simulink model "NBMS_App_Harness1"  (R2026b)
settings: Solver=FixedStepDiscrete  StopTime=25  FixedStep=0.1
undefined symbols (not defined in the file): Active_DisChrg_E, BMS_BattSoCDerate_E, BMS_BattTempDerate_E, BMS_DCDCMosfet_STS_E, BMS_HVMosfet_STS_E, BMS_MODE_E, BMS_NM_Msg_E, BMS_PMosfet_STS_E, Charger_Mode_E, Charger_Mode_Req_E, CV_Mode_Timer_E, OBC_E, VDU_MACHINE_STS_E
(part 2 of 4)

== stateflow chart NBMS_App_Harness1/Test Sequence1 ==
  state ChargeWhenIgOn
    state Run
      %% Initialize data outputs.
      AppIn_HardwiredIgn = false;
      AppIn_OBCwakeup = OBC_E.Sleep;
      AppIn_RTCwakeup = false;
      AppIn_MCUHVIL = false;
      AppIn_OBCHVIL = false;
      AppIn_SoCLEDSW = false;
      AppIn_ChgMode = Charger_Mode_E.OFF;
      AppIn_CVmodeTimer = CV_Mode_Timer_E.Off;
      AppIn_TRerror = false;
      AppIn_TRtimer = false;
      AppIn_G3CommonFlt = false;
      AppIn_G3DischargeFlt = false;
      AppIn_G4T1DischargeFlt = false;
      AppIn_G4T2DischargeFlt = false;
      AppIn_G4CommonFlt = false;
      AppIn_G4ChargeFlt = false;
      AppIn_OBCHeartbeatFail = false;
      AppIn_LoadVolt = 0;
      AppIn_PackVolt = 0;
      AppIn_ActiveDischg = Active_DisChrg_E.Inactive;
      AppIn_BattTemp = [26; 26; 26; 26; 26; 26;];
      AppIn_BattCurrent = 0;
      AppIn_BattVoltages = [4.2; 4.2; 4.2; 4.2; 4.2; 4.2; 4.2; 4.2; 4.2; 4.2; 4.2; 4.2; 4.2; 4.2; 4.2; 4.2; 4.2; 4.2; 4.2; 4.2];
      AppIn_LastStoredSOC = 0;
      AppIn_LastStoredCycle = 0;
      AppIn_I2Cerror = false;
      AppIn_LastStoredSOH = 0;
      AppIn_MachineStatus = VDU_MACHINE_STS_E.VDU_SLEEP;
      AppIn_HVMosfetfb = false;
      AppIn_DCDCMosfetfb = false;
      AppIn_PMosfetfb = false;
      AppIn_BMSVltSnsrFail = false;
      AppIn_BattPackTempSnsrFail = false;
      AppIn_VltImbFlt = false;
      AppIn_TempImbWarn = false;
      AppIn_EEPROMSoCWarn15 = false;
    state step_1
      AppIn_HardwiredIgn = true;
    state step_2
      AppIn_OBCwakeup = OBC_E.Wake_Up;
      AppIn_OBCHVIL = true;
    state step_3
      AppIn_PMosfetfb = true;
    state step_4
      AppIn_LoadVolt = 72;
      AppIn_PackVolt = 75;
    state step_5
      AppIn_HVMosfetfb = true;
    state step_6
      AppIn_DCDCMosfetfb = true;
    state step_7
      AppIn_PMosfetfb = false;
    state step_8
    (default) -> ChargeWhenIgOn.Run
    ChargeWhenIgOn.Run -> ChargeWhenIgOn.step_1 : [ after(0.1,sec) ]
    ChargeWhenIgOn.step_1 -> ChargeWhenIgOn.step_2 : [ after(0.2,sec) ]
    ChargeWhenIgOn.step_2 -> ChargeWhenIgOn.step_3 : [ after(0.5,sec) ]
    ChargeWhenIgOn.step_3 -> ChargeWhenIgOn.step_4 : [ after(0.5,sec) ]
    ChargeWhenIgOn.step_4 -> ChargeWhenIgOn.step_5 : [ after(0.1,sec) ]
    ChargeWhenIgOn.step_5 -> ChargeWhenIgOn.step_6 : [ after(0.5,sec) ]
    ChargeWhenIgOn.step_6 -> ChargeWhenIgOn.step_7 : [ after(0.5,sec) ]
    ChargeWhenIgOn.step_7 -> ChargeWhenIgOn.step_8 : [ after(0.5,sec) ]
  state DischgWhenIgOn
    state Run
      %% Initialize data outputs.
      AppIn_HardwiredIgn = false;
      AppIn_OBCwakeup = OBC_E.Sleep;
      AppIn_RTCwakeup = false;
      AppIn_MCUHVIL = false;
      AppIn_OBCHVIL = false;
      AppIn_SoCLEDSW = false;
      AppIn_ChgMode = Charger_Mode_E.OFF;
      AppIn_CVmodeTimer = CV_Mode_Timer_E.Off;
      AppIn_TRerror = false;
      AppIn_TRtimer = false;
      AppIn_G3CommonFlt = false;
      AppIn_G3DischargeFlt = false;
      AppIn_G4T1DischargeFlt = false;
      AppIn_G4T2DischargeFlt = false;
      AppIn_G4CommonFlt = false;
      AppIn_G4ChargeFlt = false;
      AppIn_OBCHeartbeatFail = false;
      AppIn_LoadVolt = 0;
      AppIn_PackVolt = 0;
      AppIn_ActiveDischg = Active_DisChrg_E.Inactive;
      AppIn_BattTemp = [26; 26; 26; 26; 26; 26;];
      AppIn_BattCurrent = 0;
      AppIn_BattVoltages = [4.2; 4.2; 4.2; 4.2; 4.2; 4.2; 4.2; 4.2; 4.2; 4.2; 4.2; 4.2; 4.2; 4.2; 4.2; 4.2; 4.2; 4.2; 4.2; 4.2];
      AppIn_LastStoredSOC = 0;
      AppIn_LastStoredCycle = 0;
      AppIn_I2Cerror = false;
      AppIn_LastStoredSOH = 0;
      AppIn_MachineStatus = VDU_MACHINE_STS_E.VDU_SLEEP;
      AppIn_HVMosfetfb = false;
      AppIn_DCDCMosfetfb = false;
      AppIn_PMosfetfb = false;
      AppIn_BMSVltSnsrFail = false;
      AppIn_BattPackTempSnsrFail = false;
      AppIn_VltImbFlt = false;
      AppIn_TempImbWarn = false;
      AppIn_EEPROMSoCWarn15 = false;
    state step_1
      AppIn_HardwiredIgn = true;
    state step_2
      AppIn_MCUHVIL  = true;
    state step_3
      AppIn_PMosfetfb = true;
    state step_4
      AppIn_LoadVolt = 72;
      AppIn_PackVolt = 75;
    state step_5
      AppIn_HVMosfetfb = true;
    state step_6
      AppIn_DCDCMosfetfb = true;
    state step_7
      AppIn_PMosfetfb = false;
    state step_8
    (default) -> DischgWhenIgOn.Run
    DischgWhenIgOn.Run -> DischgWhenIgOn.step_1 : [ true ]
    DischgWhenIgOn.step_1 -> DischgWhenIgOn.step_2 : [ after(0.2,sec) ]
    DischgWhenIgOn.step_2 -> DischgWhenIgOn.step_3 : [ after(0.5,sec) ]
    DischgWhenIgOn.step_3 -> DischgWhenIgOn.step_4 : [ after(0.5,sec) ]
    DischgWhenIgOn.step_4 -> DischgWhenIgOn.step_5 : [ after(0.2,sec) ]
    DischgWhenIgOn.step_5 -> DischgWhenIgOn.step_6 : [ after(0.5,sec) ]
    DischgWhenIgOn.step_6 -> DischgWhenIgOn.step_7 : [ after(0.5,sec) ]
    DischgWhenIgOn.step_7 -> DischgWhenIgOn.step_8 : [ after(0.5,sec) ]
  state ChargeWhenIgOff
    state Run
      %% Initialize data outputs.
      AppIn_HardwiredIgn = false;
      AppIn_OBCwakeup = OBC_E.Sleep;
      AppIn_RTCwakeup = false;
      AppIn_MCUHVIL = false;
      AppIn_OBCHVIL = false;
      AppIn_SoCLEDSW = false;
      AppIn_ChgMode = Charger_Mode_E.OFF;
      AppIn_CVmodeTimer = CV_Mode_Timer_E.Off;
      AppIn_TRerror = false;
      AppIn_TRtimer = false;
      AppIn_G3CommonFlt = false;
      AppIn_G3DischargeFlt = false;
      AppIn_G4T1DischargeFlt = false;
      AppIn_G4T2DischargeFlt = false;
      AppIn_G4CommonFlt = false;
      AppIn_G4ChargeFlt = false;
      AppIn_OBCHeartbeatFail = false;
      AppIn_LoadVolt = 0;
      AppIn_PackVolt = 0;
      AppIn_ActiveDischg = Active_DisChrg_E.Inactive;
      AppIn_BattTemp = [26; 26; 26; 26; 26; 26;];
      AppIn_BattCurrent = 0;
      AppIn_BattVoltages = [4.2; 4.2; 4.2; 4.2; 4.2; 4.2; 4.2; 4.2; 4.2; 4.2; 4.2; 4.2; 4.2; 4.2; 4.2; 4.2; 4.2; 4.2; 4.2; 4.2];
      AppIn_LastStoredSOC = 0;
      AppIn_LastStoredCycle = 0;
      AppIn_I2Cerror = false;
      AppIn_LastStoredSOH = 0;
      AppIn_MachineStatus = VDU_MACHINE_STS_E.VDU_SLEEP;
      AppIn_HVMosfetfb = false;
      AppIn_DCDCMosfetfb = false;
      AppIn_PMosfetfb = false;
      AppIn_BMSVltSnsrFail = false;
      AppIn_BattPackTempSnsrFail = false;
      AppIn_VltImbFlt = false;
      AppIn_TempImbWarn = false;
      AppIn_EEPROMSoCWarn15 = false;
    state step_1
      AppIn_OBCwakeup = OBC_E.Wake_Up;
      AppIn_OBCHVIL= true;
    state step_2
      AppIn_PMosfetfb = true;
    state step_3
      AppIn_LoadVolt = 72;
      AppIn_PackVolt = 75;
    state step_4
      AppIn_HVMosfetfb = true;
    state step_5
      AppIn_PMosfetfb = false;
    state step_6
    (default) -> ChargeWhenIgOff.Run
    ChargeWhenIgOff.Run -> ChargeWhenIgOff.step_1
    ChargeWhenIgOff.step_1 -> ChargeWhenIgOff.step_2 : [ after(0.5,sec) ]
    ChargeWhenIgOff.step_2 -> ChargeWhenIgOff.step_3 : [ after(0.5,sec) ]
    ChargeWhenIgOff.step_3 -> ChargeWhenIgOff.step_4 : [ after(0.5,sec) ]
    ChargeWhenIgOff.step_4 -> ChargeWhenIgOff.step_5 : [ after(0.5,sec) ]
    ChargeWhenIgOff.step_5 -> ChargeWhenIgOff.step_6 : [ after(0.5,sec) ]
  state ChgToDischgIgOn
    state Run
      %% Initialize data outputs.
      AppIn_HardwiredIgn = false;
      AppIn_OBCwakeup = OBC_E.Sleep;
      AppIn_RTCwakeup = false;
      AppIn_MCUHVIL = false;
      AppIn_OBCHVIL = false;
      AppIn_SoCLEDSW = false;
      AppIn_ChgMode = Charger_Mode_E.OFF;
      AppIn_CVmodeTimer = CV_Mode_Timer_E.Off;
      AppIn_TRerror = false;
      AppIn_TRtimer = false;
      AppIn_G3CommonFlt = false;
      AppIn_G3DischargeFlt = false;
      AppIn_G4T1DischargeFlt = false;
      AppIn_G4T2DischargeFlt = false;
      AppIn_G4CommonFlt = false;
      AppIn_G4ChargeFlt = false;
      AppIn_OBCHeartbeatFail = false;
      AppIn_LoadVolt = 0;
      AppIn_PackVolt = 0;
      AppIn_ActiveDischg = Active_DisChrg_E.Inactive;
      AppIn_BattTemp = [26; 26; 26; 26; 26; 26;];
      AppIn_BattCurrent = 0;
      AppIn_BattVoltages = [4.2; 4.2; 4.2; 4.2; 4.2; 4.2; 4.2; 4.2; 4.2; 4.2; 4.2; 4.2; 4.2; 4.2; 4.2; 4.2; 4.2; 4.2; 4.2; 4.2];
      AppIn_LastStoredSOC = 0;
      AppIn_LastStoredCycle = 0;
      AppIn_I2Cerror = false;
      AppIn_LastStoredSOH = 0;
      AppIn_MachineStatus = VDU_MACHINE_STS_E.VDU_SLEEP;
      AppIn_HVMosfetfb = false;
      AppIn_DCDCMosfetfb = false;
      AppIn_PMosfetfb = false;
      AppIn_BMSVltSnsrFail = false;
      AppIn_BattPackTempSnsrFail = false;
      AppIn_VltImbFlt = false;
      AppIn_TempImbWarn = false;
      AppIn_EEPROMSoCWarn15 = false;
    state step_1
      AppIn_HardwiredIgn = true;
    state step_2
      AppIn_OBCwakeup = OBC_E.Wake_Up;
      AppIn_OBCHVIL= true;
    state step_3
      AppIn_PMosfetfb = true;
    state step_4
      AppIn_LoadVolt = 72;
      AppIn_PackVolt = 75;
    state step_5
      AppIn_HVMosfetfb = true;
    state step_6
      AppIn_DCDCMosfetfb = true;
    state step_7
      AppIn_PMosfetfb = false;
    state step_8
    state step_9
      AppIn_OBCHVIL= false;
    state step_10
      AppIn_MCUHVIL  = true;
    state step_11
    (default) -> ChgToDischgIgOn.Run
    ChgToDischgIgOn.Run -> ChgToDischgIgOn.step_1
    ChgToDischgIgOn.step_1 -> ChgToDischgIgOn.step_2 : [ after(0.2,sec) ]
    ChgToDischgIgOn.step_2 -> ChgToDischgIgOn.step_3 : [ after(0.5,sec) ]
    ChgToDischgIgOn.step_3 -> ChgToDischgIgOn.step_4 : [ after(0.5,sec) ]
    ChgToDischgIgOn.step_4 -> ChgToDischgIgOn.step_5 : [ after(0.2,sec) ]
    ChgToDischgIgOn.step_5 -> ChgToDischgIgOn.step_6 : [ after(0.5,sec) ]
    ChgToDischgIgOn.step_6 -> ChgToDischgIgOn.step_7 : [ after(0.5,sec) ]
    ChgToDischgIgOn.step_7 -> ChgToDischgIgOn.step_8 : [ after(0.5,sec) ]
    ChgToDischgIgOn.step_8 -> ChgToDischgIgOn.step_9 : [ after(1,sec) ]
    ChgToDischgIgOn.step_9 -> ChgToDischgIgOn.step_10 : [ after(0.2,sec) ]
    ChgToDischgIgOn.step_10 -> ChgToDischgIgOn.step_11 : [ after(0.5,sec) ]
  state SleepToStandby
    state Run
      %% Initialize data outputs.
      AppIn_HardwiredIgn = false;
      AppIn_OBCwakeup = OBC_E.Sleep;
      AppIn_RTCwakeup = false;
      AppIn_MCUHVIL = false;
      AppIn_OBCHVIL = false;
      AppIn_SoCLEDSW = false;
      AppIn_ChgMode = Charger_Mode_E.OFF;
      AppIn_CVmodeTimer = CV_Mode_Timer_E.Off;
      AppIn_TRerror = false;
      AppIn_TRtimer = false;
      AppIn_G3CommonFlt = false;
      AppIn_G3DischargeFlt = false;
      AppIn_G4T1DischargeFlt = false;
      AppIn_G4T2DischargeFlt = false;
      AppIn_G4CommonFlt = false;
      AppIn_G4ChargeFlt = false;
      AppIn_OBCHeartbeatFail = false;
      AppIn_LoadVolt = 0;
      AppIn_PackVolt = 0;
      AppIn_ActiveDischg = Active_DisChrg_E.Inactive;
      AppIn_BattTemp = [26; 26; 26; 26; 26; 26;];
      AppIn_BattCurrent = 0;
      AppIn_BattVoltages = [4.2; 4.2; 4.2; 4.2; 4.2; 4.2; 4.2; 4.2; 4.2; 4.2; 4.2; 4.2; 4.2; 4.2; 4.2; 4.2; 4.2; 4.2; 4.2; 4.2];
      AppIn_LastStoredSOC = 0;
      AppIn_LastStoredCycle = 0;
      AppIn_I2Cerror = false;
      AppIn_LastStoredSOH = 0;
      AppIn_MachineStatus = VDU_MACHINE_STS_E.VDU_SLEEP;
      AppIn_HVMosfetfb = false;
      AppIn_DCDCMosfetfb = false;
      AppIn_PMosfetfb = false;
      AppIn_BMSVltSnsrFail = false;
      AppIn_BattPackTempSnsrFail = false;
      AppIn_VltImbFlt = false;
      AppIn_TempImbWarn = false;
      AppIn_EEPROMSoCWarn15 = false;
    state step_1
      AppIn_HardwiredIgn = true;
    state step_2
    (default) -> SleepToStandby.Run
    SleepToStandby.Run -> SleepToStandby.step_1
    SleepToStandby.step_1 -> SleepToStandby.step_2 : [ after(1,sec) ]
  state DischgToStandby
    state Run
      %% Initialize data outputs.
      AppIn_HardwiredIgn = false;
      AppIn_OBCwakeup = OBC_E.Sleep;
      AppIn_RTCwakeup = false;
      AppIn_MCUHVIL = false;
      AppIn_OBCHVIL = false;
      AppIn_SoCLEDSW = false;
      AppIn_ChgMode = Charger_Mode_E.OFF;
      AppIn_CVmodeTimer = CV_Mode_Timer_E.Off;
      AppIn_TRerror = false;
      AppIn_TRtimer = false;
      AppIn_G3CommonFlt = false;
      AppIn_G3DischargeFlt = false;
      AppIn_G4T1DischargeFlt = false;
      AppIn_G4T2DischargeFlt = false;
      AppIn_G4CommonFlt = false;
      AppIn_G4ChargeFlt = false;
      AppIn_OBCHeartbeatFail = false;
      AppIn_LoadVolt = 0;
      AppIn_PackVolt = 0;
      AppIn_ActiveDischg = Active_DisChrg_E.Inactive;
      AppIn_BattTemp = [26; 26; 26; 26; 26; 26;];
      AppIn_BattCurrent = 0;
      AppIn_BattVoltages = [4.2; 4.2; 4.2; 4.2; 4.2; 4.2; 4.2; 4.2; 4.2; 4.2; 4.2; 4.2; 4.2; 4.2; 4.2; 4.2; 4.2; 4.2; 4.2; 4.2];
      AppIn_LastStoredSOC = 0;
      AppIn_LastStoredCycle = 0;
      AppIn_I2Cerror = false;
      AppIn_LastStoredSOH = 0;
      AppIn_MachineStatus = VDU_MACHINE_STS_E.VDU_SLEEP;
      AppIn_HVMosfetfb = false;
      AppIn_DCDCMosfetfb = false;
      AppIn_PMosfetfb = false;
      AppIn_BMSVltSnsrFail = false;
      AppIn_BattPackTempSnsrFail = false;
      AppIn_VltImbFlt = false;
      AppIn_TempImbWarn = false;
      AppIn_EEPROMSoCWarn15 = false;
    state step_1
      AppIn_HardwiredIgn = true;
    state step_2
      AppIn_MCUHVIL  = true;
    state step_3
      AppIn_PMosfetfb = true;
    state step_4
      AppIn_LoadVolt = 72;
      AppIn_PackVolt = 75;
    state step_5
      AppIn_HVMosfetfb = true;
    state step_6
      AppIn_DCDCMosfetfb = true;
    state step_7
      AppIn_PMosfetfb = false;
    state step_8
    state step_9
      AppIn_HardwiredIgn = false;
    state step_10
      AppIn_HVMosfetfb = false;
    state step_11
    (default) -> DischgToStandby.Run
    DischgToStandby.Run -> DischgToStandby.step_1
    DischgToStandby.step_1 -> DischgToStandby.step_2 : [ after(0.2,sec) ]
    DischgToStandby.step_2 -> DischgToStandby.step_3 : [ after(0.2,sec) ]
    DischgToStandby.step_3 -> DischgToStandby.step_4 : [ after(0.3,sec) ]
    DischgToStandby.step_4 -> DischgToStandby.step_5 : [ after(0.2,sec) ]
    DischgToStandby.step_5 -> DischgToStandby.step_6 : [ after(0.3,sec) ]
    DischgToStandby.step_6 -> DischgToStandby.step_7 : [ after(0.3,sec) ]
    DischgToStandby.step_7 -> DischgToStandby.step_8 : [ after(0.3,sec) ]
    DischgToStandby.step_8 -> DischgToStandby.step_9 : [ after(1,sec) ]
    DischgToStandby.step_9 -> DischgToStandby.step_10 : [ after(0.3,sec) ]
    DischgToStandby.step_10 -> DischgToStandby.step_11 : [ after(0.5,sec) ]
  state StandbyToDischgIgOn
    state Run
      %% Initialize data outputs.
      AppIn_HardwiredIgn = false;
      AppIn_OBCwakeup = OBC_E.Sleep;
      AppIn_RTCwakeup = false;
      AppIn_MCUHVIL = false;
      AppIn_OBCHVIL = false;
      AppIn_SoCLEDSW = false;
      AppIn_ChgMode = Charger_Mode_E.OFF;
      AppIn_CVmodeTimer = CV_Mode_Timer_E.Off;
      AppIn_TRerror = false;
      AppIn_TRtimer = false;
      AppIn_G3CommonFlt = false;
      AppIn_G3DischargeFlt = false;
      AppIn_G4T1DischargeFlt = false;
      AppIn_G4T2DischargeFlt = false;
      AppIn_G4CommonFlt = false;
      AppIn_G4ChargeFlt = false;
      AppIn_OBCHeartbeatFail = false;
      AppIn_LoadVolt = 0;
      AppIn_PackVolt = 0;
      AppIn_ActiveDischg = Active_DisChrg_E.Inactive;
      AppIn_BattTemp = [26; 26; 26; 26; 26; 26;];
      AppIn_BattCurrent = 0;
      AppIn_BattVoltages = [4.2; 4.2; 4.2; 4.2; 4.2; 4.2; 4.2; 4.2; 4.2; 4.2; 4.2; 4.2; 4.2; 4.2; 4.2; 4.2; 4.2; 4.2; 4.2; 4.2];
      AppIn_LastStoredSOC = 0;
      AppIn_LastStoredCycle = 0;
      AppIn_I2Cerror = false;
      AppIn_LastStoredSOH = 0;
      AppIn_MachineStatus = VDU_MACHINE_STS_E.VDU_SLEEP;
      AppIn_HVMosfetfb = false;
      AppIn_DCDCMosfetfb = false;
      AppIn_PMosfetfb = false;
      AppIn_BMSVltSnsrFail = false;
      AppIn_BattPackTempSnsrFail = false;
      AppIn_VltImbFlt = false;
      AppIn_TempImbWarn = false;
      AppIn_EEPROMSoCWarn15 = false;
    state step_1
      AppIn_HardwiredIgn = true;
    state step_2
      AppIn_OBCwakeup = OBC_E.Wake_Up;
      AppIn_OBCHVIL= true;
    state step_3
      AppIn_PMosfetfb = true;
    state step_4
      AppIn_LoadVolt = 72;
      AppIn_PackVolt = 75;
    state step_5
      AppIn_HVMosfetfb = true;
    state step_6
      AppIn_DCDCMosfetfb = true;
    state step_7
      AppIn_PMosfetfb = false;
    state step_8
    state step_9
      AppIn_OBCwakeup = OBC_E.Sleep;
      AppIn_OBCHVIL= false;
    state step_10
    state step_11
      AppIn_HVMosfetfb = false;
    state step_12
      AppIn_MCUHVIL  = true;
    state step_13
      AppIn_PMosfetfb = true;
    state step_14
      AppIn_HVMosfetfb = true;
    state step_15
      AppIn_PMosfetfb = false;
    state step_16
    (default) -> StandbyToDischgIgOn.Run
    StandbyToDischgIgOn.Run -> StandbyToDischgIgOn.step_1
    StandbyToDischgIgOn.step_1 -> StandbyToDischgIgOn.step_2 : [ after(0.2,sec) ]
    StandbyToDischgIgOn.step_2 -> StandbyToDischgIgOn.step_3 : [ after(0.2,sec) ]
    StandbyToDischgIgOn.step_3 -> StandbyToDischgIgOn.step_4 : [ after(0.3,sec) ]
    StandbyToDischgIgOn.step_4 -> StandbyToDischgIgOn.step_5 : [ after(0.2,sec) ]
    StandbyToDischgIgOn.step_5 -> StandbyToDischgIgOn.step_6 : [ after(0.3,sec) ]
    StandbyToDischgIgOn.step_6 -> StandbyToDischgIgOn.step_7 : [ after(0.3,sec) ]
    StandbyToDischgIgOn.step_7 -> StandbyToDischgIgOn.step_8 : [ after(0.3,sec) ]
    StandbyToDischgIgOn.step_8 -> StandbyToDischgIgOn.step_9 : [ after(1,sec) ]
    StandbyToDischgIgOn.step_9 -> StandbyToDischgIgOn.step_10 : [ after(0.3,sec) ]
    StandbyToDischgIgOn.step_10 -> StandbyToDischgIgOn.step_11 : [ after(1,sec) ]
    StandbyToDischgIgOn.step_11 -> StandbyToDischgIgOn.step_12 : [ after(0.5,sec) ]
    StandbyToDischgIgOn.step_12 -> StandbyToDischgIgOn.step_13 : [ after(0.2,sec) ]
    StandbyToDischgIgOn.step_13 -> StandbyToDischgIgOn.step_14 : [ after(0.5,sec) ]
    StandbyToDischgIgOn.step_14 -> StandbyToDischgIgOn.step_15 : [ after(0.5,sec) ]
    StandbyToDischgIgOn.step_15 -> StandbyToDischgIgOn.step_16 : [ after(1,sec) ]
  state IgOffToOnInCharge
    state Run
      %% Initialize data outputs.
      AppIn_HardwiredIgn = false;
      AppIn_OBCwakeup = OBC_E.Sleep;
      AppIn_RTCwakeup = false;
      AppIn_MCUHVIL = false;
      AppIn_OBCHVIL = false;
      AppIn_SoCLEDSW = false;
      AppIn_ChgMode = Charger_Mode_E.OFF;
      AppIn_CVmodeTimer = CV_Mode_Timer_E.Off;
      AppIn_TRerror = false;
      AppIn_TRtimer = false;
      AppIn_G3CommonFlt = false;
      AppIn_G3DischargeFlt = false;
      AppIn_G4T1DischargeFlt = false;
      AppIn_G4T2DischargeFlt = false;
      AppIn_G4CommonFlt = false;
      AppIn_G4ChargeFlt = false;
      AppIn_OBCHeartbeatFail = false;
      AppIn_LoadVolt = 0;
      AppIn_PackVolt = 0;
      AppIn_ActiveDischg = Active_DisChrg_E.Inactive;
      AppIn_BattTemp = [26; 26; 26; 26; 26; 26;];
      AppIn_BattCurrent = 0;
      AppIn_BattVoltages = [4.2; 4.2; 4.2; 4.2; 4.2; 4.2; 4.2; 4.2; 4.2; 4.2; 4.2; 4.2; 4.2; 4.2; 4.2; 4.2; 4.2; 4.2; 4.2; 4.2];
      AppIn_LastStoredSOC = 0;
      AppIn_LastStoredCycle = 0;
      AppIn_I2Cerror = false;
      AppIn_LastStoredSOH = 0;
      AppIn_MachineStatus = VDU_MACHINE_STS_E.VDU_SLEEP;
      AppIn_HVMosfetfb = false;
      AppIn_DCDCMosfetfb = false;
      AppIn_PMosfetfb = false;
      AppIn_BMSVltSnsrFail = false;
      AppIn_BattPackTempSnsrFail = false;
      AppIn_VltImbFlt = false;
      AppIn_TempImbWarn = false;
      AppIn_EEPROMSoCWarn15 = false;
    state step_1
      AppIn_OBCwakeup = OBC_E.Wake_Up;
      AppIn_OBCHVIL= true;
    state step_2
      AppIn_PMosfetfb = true;
    state step_3
      AppIn_LoadVolt = 72;
      AppIn_PackVolt = 75;
    state step_4
      AppIn_HVMosfetfb = true;
    state step_5
      AppIn_PMosfetfb = false;
    state step_6
    state step_7
      AppIn_HardwiredIgn = true;
    state step_8
    (default) -> IgOffToOnInCharge.Run
    IgOffToOnInCharge.Run -> IgOffToOnInCharge.step_1
    IgOffToOnInCharge.step_1 -> IgOffToOnInCharge.step_2 : [ after(0.2,sec) ]
    IgOffToOnInCharge.step_2 -> IgOffToOnInCharge.step_3 : [ after(0.3,sec) ]
    IgOffToOnInCharge.step_3 -> IgOffToOnInCharge.step_4 : [ after(0.2,sec) ]
    IgOffToOnInCharge.step_4 -> IgOffToOnInCharge.step_5 : [ after(0.5,sec) ]
    IgOffToOnInCharge.step_5 -> IgOffToOnInCharge.step_6 : [ after(0.3,sec) ]
    IgOffToOnInCharge.step_7 -> IgOffToOnInCharge.step_8 : [ after(0.2,sec) ]
    IgOffToOnInCharge.step_6 -> IgOffToOnInCharge.step_7 : [ after(1,sec) ]
  state IgOnToOffInCharge
    state Run
      %% Initialize data outputs.
      AppIn_HardwiredIgn = false;
      AppIn_OBCwakeup = OBC_E.Sleep;
      AppIn_RTCwakeup = false;
      AppIn_MCUHVIL = false;
      AppIn_OBCHVIL = false;
      AppIn_SoCLEDSW = false;
      AppIn_ChgMode = Charger_Mode_E.OFF;
      AppIn_CVmodeTimer = CV_Mode_Timer_E.Off;
      AppIn_TRerror = false;
      AppIn_TRtimer = false;
      AppIn_G3CommonFlt = false;
      AppIn_G3DischargeFlt = false;
      AppIn_G4T1DischargeFlt = false;
      AppIn_G4T2DischargeFlt = false;
      AppIn_G4CommonFlt = false;
      AppIn_G4ChargeFlt = false;
      AppIn_OBCHeartbeatFail = false;
      AppIn_LoadVolt = 0;
      AppIn_PackVolt = 0;
      AppIn_ActiveDischg = Active_DisChrg_E.Inactive;
      AppIn_BattTemp = [26; 26; 26; 26; 26; 26;];
      AppIn_BattCurrent = 0;
      AppIn_BattVoltages = [4.2; 4.2; 4.2; 4.2; 4.2; 4.2; 4.2; 4.2; 4.2; 4.2; 4.2; 4.2; 4.2; 4.2; 4.2; 4.2; 4.2; 4.2; 4.2; 4.2];
      AppIn_LastStoredSOC = 0;
      AppIn_LastStoredCycle = 0;
      AppIn_I2Cerror = false;
      AppIn_LastStoredSOH = 0;
      AppIn_MachineStatus = VDU_MACHINE_STS_E.VDU_SLEEP;
      AppIn_HVMosfetfb = false;
      AppIn_DCDCMosfetfb = false;
      AppIn_PMosfetfb = false;
      AppIn_BMSVltSnsrFail = false;
      AppIn_BattPackTempSnsrFail = false;
      AppIn_VltImbFlt = false;
      AppIn_TempImbWarn = false;
      AppIn_EEPROMSoCWarn15 = false;
    state step_1
      AppIn_HardwiredIgn = true;
    state step_2
      AppIn_OBCwakeup = OBC_E.Wake_Up;
      AppIn_OBCHVIL= true;
    state step_3
      AppIn_PMosfetfb = true;
    state step_4
      AppIn_LoadVolt = 72;
      AppIn_PackVolt = 75;
    state step_5
      AppIn_HVMosfetfb = true;
    state step_6
      AppIn_DCDCMosfetfb = true;
    state step_7
      AppIn_PMosfetfb = false;
    state step_8
    state step_9
      AppIn_HardwiredIgn = false;
    state step_10
      AppIn_ActiveDischg = Active_DisChrg_E.Completed;
    (default) -> IgOnToOffInCharge.Run
    IgOnToOffInCharge.Run -> IgOnToOffInCharge.step_1
    IgOnToOffInCharge.step_1 -> IgOnToOffInCharge.step_2 : [ after(0.2,sec) ]
    IgOnToOffInCharge.step_2 -> IgOnToOffInCharge.step_3 : [ after(0.2,sec) ]
    IgOnToOffInCharge.step_3 -> IgOnToOffInCharge.step_4 : [ after(0.3,sec) ]
    IgOnToOffInCharge.step_4 -> IgOnToOffInCharge.step_5 : [ after(0.2,sec) ]
    IgOnToOffInCharge.step_5 -> IgOnToOffInCharge.step_6 : [ after(0.3,sec) ]
    IgOnToOffInCharge.step_6 -> IgOnToOffInCharge.step_7 : [ after(0.3,sec) ]
    IgOnToOffInCharge.step_7 -> IgOnToOffInCharge.step_8 : [ after(0.3,sec) ]
    IgOnToOffInCharge.step_8 -> IgOnToOffInCharge.step_9 : [ after(1,sec) ]
    IgOnToOffInCharge.step_9 -> IgOnToOffInCharge.step_10 : [ after(0.3,sec) ]
  state VehPoweredOff
    state Run
      %% Initialize data outputs.
      AppIn_HardwiredIgn = false;
      AppIn_OBCwakeup = OBC_E.Sleep;
      AppIn_RTCwakeup = false;
      AppIn_MCUHVIL = false;
      AppIn_OBCHVIL = false;
      AppIn_SoCLEDSW = false;
      AppIn_ChgMode = Charger_Mode_E.OFF;
      AppIn_CVmodeTimer = CV_Mode_Timer_E.Off;
      AppIn_TRerror = false;
      AppIn_TRtimer = false;
      AppIn_G3CommonFlt = false;
      AppIn_G3DischargeFlt = false;
      AppIn_G4T1DischargeFlt = false;
      AppIn_G4T2DischargeFlt = false;
      AppIn_G4CommonFlt = false;
      AppIn_G4ChargeFlt = false;
      AppIn_OBCHeartbeatFail = false;
      AppIn_LoadVolt = 0;
      AppIn_PackVolt = 0;
      AppIn_ActiveDischg = Active_DisChrg_E.Inactive;
      AppIn_BattTemp = [26; 26; 26; 26; 26; 26;];
      AppIn_BattCurrent = 0;
      AppIn_BattVoltages = [4.2; 4.2; 4.2; 4.2; 4.2; 4.2; 4.2; 4.2; 4.2; 4.2; 4.2; 4.2; 4.2; 4.2; 4.2; 4.2; 4.2; 4.2; 4.2; 4.2];
      AppIn_LastStoredSOC = 0;
      AppIn_LastStoredCycle = 0;
      AppIn_I2Cerror = false;
      AppIn_LastStoredSOH = 0;
      AppIn_MachineStatus = VDU_MACHINE_STS_E.VDU_SLEEP;
      AppIn_HVMosfetfb = false;
      AppIn_DCDCMosfetfb = false;
      AppIn_PMosfetfb = false;
      AppIn_BMSVltSnsrFail = false;
      AppIn_BattPackTempSnsrFail = false;
      AppIn_VltImbFlt = false;
      AppIn_TempImbWarn = false;
      AppIn_EEPROMSoCWarn15 = false;
    state step_1
      AppIn_HardwiredIgn = true;
    state step_2
      AppIn_MCUHVIL  = true;
    state step_3
      AppIn_PMosfetfb = true;
    state step_4
      AppIn_LoadVolt = 72;
      AppIn_PackVolt = 75;
    state step_5
      AppIn_HVMosfetfb = true;
    state step_6
      AppIn_DCDCMosfetfb = true;
    state step_7
      AppIn_PMosfetfb = false;
    state step_8
    state step_9
      AppIn_HardwiredIgn = false;
    state step_10
      AppIn_HVMosfetfb = false;
    state step_11
      AppIn_ActiveDischg = Active_DisChrg_E.Completed;
    state step_12
    (default) -> VehPoweredOff.Run
    VehPoweredOff.Run -> VehPoweredOff.step_1
    VehPoweredOff.step_1 -> VehPoweredOff.step_2 : [ after(0.2,sec) ]
    VehPoweredOff.step_2 -> VehPoweredOff.step_3 : [ after(0.2,sec) ]
    VehPoweredOff.step_3 -> VehPoweredOff.step_4 : [ after(0.3,sec) ]
    VehPoweredOff.step_4 -> VehPoweredOff.step_5 : [ after(0.2,sec) ]
    VehPoweredOff.step_5 -> VehPoweredOff.step_6 : [ after(0.3,sec) ]
    VehPoweredOff.step_6 -> VehPoweredOff.step_7 : [ after(0.3,sec) ]
    VehPoweredOff.step_7 -> VehPoweredOff.step_8 : [ after(0.3,sec) ]
    VehPoweredOff.step_8 -> VehPoweredOff.step_9 : [ after(1,sec) ]
    VehPoweredOff.step_9 -> VehPoweredOff.step_10 : [ after(0.3,sec) ]
    VehPoweredOff.step_10 -> VehPoweredOff.step_11 : [ after(0.3,sec) ]
    VehPoweredOff.step_11 -> VehPoweredOff.step_12 : [ after(0.3,sec) ]
  state G4T1DischgFlt
    state Run
      %% Initialize data outputs.
      AppIn_HardwiredIgn = false;
      AppIn_OBCwakeup = OBC_E.Sleep;
      AppIn_RTCwakeup = false;
      AppIn_MCUHVIL = false;
      AppIn_OBCHVIL = false;
      AppIn_SoCLEDSW = false;
      AppIn_ChgMode = Charger_Mode_E.OFF;
      AppIn_CVmodeTimer = CV_Mode_Timer_E.Off;
      AppIn_TRerror = false;
      AppIn_TRtimer = false;
      AppIn_G3CommonFlt = false;
      AppIn_G3DischargeFlt = false;
      AppIn_G4T1DischargeFlt = false;
      AppIn_G4T2DischargeFlt = false;
      AppIn_G4CommonFlt = false;
      AppIn_G4ChargeFlt = false;
      AppIn_OBCHeartbeatFail = false;
      AppIn_LoadVolt = 0;
      AppIn_PackVolt = 0;
      AppIn_ActiveDischg = Active_DisChrg_E.Inactive;
      AppIn_BattTemp = [26; 26; 26; 26; 26; 26;];
      AppIn_BattCurrent = 0;
      AppIn_BattVoltages = [4.2; 4.2; 4.2; 4.2; 4.2; 4.2; 4.2; 4.2; 4.2; 4.2; 4.2; 4.2; 4.2; 4.2; 4.2; 4.2; 4.2; 4.2; 4.2; 4.2];
      AppIn_LastStoredSOC = 0;
      AppIn_LastStoredCycle = 0;
      AppIn_I2Cerror = false;
      AppIn_LastStoredSOH = 0;
      AppIn_MachineStatus = VDU_MACHINE_STS_E.VDU_SLEEP;
      AppIn_HVMosfetfb = false;
      AppIn_DCDCMosfetfb = false;
      AppIn_PMosfetfb = false;
      AppIn_BMSVltSnsrFail = false;
      AppIn_BattPackTempSnsrFail = false;
      AppIn_VltImbFlt = false;
      AppIn_TempImbWarn = false;
      AppIn_EEPROMSoCWarn15 = false;
    state step_1
      AppIn_HardwiredIgn = true;
    state step_2
      AppIn_MCUHVIL  = true;
    state step_3
      AppIn_PMosfetfb = true;
    state step_4
      AppIn_LoadVolt = 72;
      AppIn_PackVolt = 75;
    state step_5
      AppIn_HVMosfetfb = true;
    state step_6
      AppIn_DCDCMosfetfb = true;
    state step_7
      AppIn_PMosfetfb = false;
    state step_8
    state step_9
      AppIn_G4T1DischargeFlt = true;
    state step_10
    (default) -> G4T1DischgFlt.Run
    G4T1DischgFlt.Run -> G4T1DischgFlt.step_1
    G4T1DischgFlt.step_1 -> G4T1DischgFlt.step_2 : [ after(0.2,sec) ]
    G4T1DischgFlt.step_2 -> G4T1DischgFlt.step_3 : [ after(0.2,sec) ]
    G4T1DischgFlt.step_3 -> G4T1DischgFlt.step_4 : [ after(0.3,sec) ]
    G4T1DischgFlt.step_4 -> G4T1DischgFlt.step_5 : [ after(0.2,sec) ]
    G4T1DischgFlt.step_5 -> G4T1DischgFlt.step_6 : [ after(0.3,sec) ]
    G4T1DischgFlt.step_6 -> G4T1DischgFlt.step_7 : [ after(0.3,sec) ]
    G4T1DischgFlt.step_7 -> G4T1DischgFlt.step_8 : [ after(0.3,sec) ]
    G4T1DischgFlt.step_8 -> G4T1DischgFlt.step_9 : [ after(1,sec) ]
    G4T1DischgFlt.step_9 -> G4T1DischgFlt.step_10 : [ after(6,sec) ]
  state G4T2DischgFlt
    state Run
      %% Initialize data outputs.
      AppIn_HardwiredIgn = false;
      AppIn_OBCwakeup = OBC_E.Sleep;
      AppIn_RTCwakeup = false;
      AppIn_MCUHVIL = false;
      AppIn_OBCHVIL = false;
      AppIn_SoCLEDSW = false;
      AppIn_ChgMode = Charger_Mode_E.OFF;
      AppIn_CVmodeTimer = CV_Mode_Timer_E.Off;
      AppIn_TRerror = false;
      AppIn_TRtimer = false;
      AppIn_G3CommonFlt = false;
      AppIn_G3DischargeFlt = false;
      AppIn_G4T1DischargeFlt = false;
      AppIn_G4T2DischargeFlt = false;
      AppIn_G4CommonFlt = false;
      AppIn_G4ChargeFlt = false;
      AppIn_OBCHeartbeatFail = false;
      AppIn_LoadVolt = 0;
      AppIn_PackVolt = 0;
      AppIn_ActiveDischg = Active_DisChrg_E.Inactive;
      AppIn_BattTemp = [26; 26; 26; 26; 26; 26;];
      AppIn_BattCurrent = 0;
      AppIn_BattVoltages = [4.2; 4.2; 4.2; 4.2; 4.2; 4.2; 4.2; 4.2; 4.2; 4.2; 4.2; 4.2; 4.2; 4.2; 4.2; 4.2; 4.2; 4.2; 4.2; 4.2];
      AppIn_LastStoredSOC = 0;
      AppIn_LastStoredCycle = 0;
      AppIn_I2Cerror = false;
      AppIn_LastStoredSOH = 0;
      AppIn_MachineStatus = VDU_MACHINE_STS_E.VDU_SLEEP;
      AppIn_HVMosfetfb = false;
      AppIn_DCDCMosfetfb = false;
      AppIn_PMosfetfb = false;
      AppIn_BMSVltSnsrFail = false;
      AppIn_BattPackTempSnsrFail = false;
      AppIn_VltImbFlt = false;
      AppIn_TempImbWarn = false;
      AppIn_EEPROMSoCWarn15 = false;
    state step_1
      AppIn_HardwiredIgn = true;
    state step_2
      AppIn_MCUHVIL  = true;
    state step_3
      AppIn_PMosfetfb = true;
    state step_4
      AppIn_LoadVolt = 72;
      AppIn_PackVolt = 75;
    state step_5
      AppIn_HVMosfetfb = true;
    state step_6
      AppIn_DCDCMosfetfb = true;
    state step_7
      AppIn_PMosfetfb = false;
    state step_8
    state step_9
      AppIn_G4T2DischargeFlt = true;
    state step_10
    (default) -> G4T2DischgFlt.Run
    G4T2DischgFlt.Run -> G4T2DischgFlt.step_1
    G4T2DischgFlt.step_1 -> G4T2DischgFlt.step_2 : [ after(0.2,sec) ]
    G4T2DischgFlt.step_2 -> G4T2DischgFlt.step_3 : [ after(0.2,sec) ]
    G4T2DischgFlt.step_3 -> G4T2DischgFlt.step_4 : [ after(0.3,sec) ]
    G4T2DischgFlt.step_4 -> G4T2DischgFlt.step_5 : [ after(0.2,sec) ]
    G4T2DischgFlt.step_5 -> G4T2DischgFlt.step_6 : [ after(0.3,sec) ]
    G4T2DischgFlt.step_6 -> G4T2DischgFlt.step_7 : [ after(0.3,sec) ]
    G4T2DischgFlt.step_7 -> G4T2DischgFlt.step_8 : [ after(0.3,sec) ]
    G4T2DischgFlt.step_8 -> G4T2DischgFlt.step_9 : [ after(1,sec) ]
    G4T2DischgFlt.step_9 -> G4T2DischgFlt.step_10 : [ after(6,sec) ]
  state G4CommonFlt
    state Run
      %% Initialize data outputs.
      AppIn_HardwiredIgn = false;
      AppIn_OBCwakeup = OBC_E.Sleep;
      AppIn_RTCwakeup = false;
      AppIn_MCUHVIL = false;
      AppIn_OBCHVIL = false;
      AppIn_SoCLEDSW = false;
      AppIn_ChgMode = Charger_Mode_E.OFF;
      AppIn_CVmodeTimer = CV_Mode_Timer_E.Off;
      AppIn_TRerror = false;
      AppIn_TRtimer = false;
      AppIn_G3CommonFlt = false;
      AppIn_G3DischargeFlt = false;
      AppIn_G4T1DischargeFlt = false;
      AppIn_G4T2DischargeFlt = false;
      AppIn_G4CommonFlt = false;
      AppIn_G4ChargeFlt = false;
      AppIn_OBCHeartbeatFail = false;
      AppIn_LoadVolt = 0;
      AppIn_PackVolt = 0;
      AppIn_ActiveDischg = Active_DisChrg_E.Inactive;
      AppIn_BattTemp = [26; 26; 26; 26; 26; 26;];
      AppIn_BattCurrent = 0;
      AppIn_BattVoltages = [4.2; 4.2; 4.2; 4.2; 4.2; 4.2; 4.2; 4.2; 4.2; 4.2; 4.2; 4.2; 4.2; 4.2; 4.2; 4.2; 4.2; 4.2; 4.2; 4.2];
      AppIn_LastStoredSOC = 0;
      AppIn_LastStoredCycle = 0;
      AppIn_I2Cerror = false;
      AppIn_LastStoredSOH = 0;
      AppIn_MachineStatus = VDU_MACHINE_STS_E.VDU_SLEEP;
      AppIn_HVMosfetfb = false;
      AppIn_DCDCMosfetfb = false;
      AppIn_PMosfetfb = false;
      AppIn_BMSVltSnsrFail = false;
      AppIn_BattPackTempSnsrFail = false;
      AppIn_VltImbFlt = false;
      AppIn_TempImbWarn = false;
      AppIn_EEPROMSoCWarn15 = false;
    state step_1
      AppIn_HardwiredIgn = true;
    state step_2
      AppIn_MCUHVIL  = true;
    state step_3
      AppIn_PMosfetfb = true;
    state step_4
      AppIn_LoadVolt = 72;
      AppIn_PackVolt = 75;
    state step_5
      AppIn_HVMosfetfb = true;
    state step_6
      AppIn_DCDCMosfetfb = true;
    state step_7
      AppIn_PMosfetfb = false;
    state step_8
    state step_9
      AppIn_G4CommonFlt = true;
    state step_10
    G4CommonFlt.step_1 -> G4CommonFlt.step_2 : [ after(0.2,sec) ]
    G4CommonFlt.step_2 -> G4CommonFlt.step_3 : [ after(0.2,sec) ]
    G4CommonFlt.step_3 -> G4CommonFlt.step_4 : [ after(0.3,sec) ]
    G4CommonFlt.step_4 -> G4CommonFlt.step_5 : [ after(0.2,sec) ]
    G4CommonFlt.step_5 -> G4CommonFlt.step_6 : [ after(0.3,sec) ]
    G4CommonFlt.step_6 -> G4CommonFlt.step_7 : [ after(0.3,sec) ]
    G4CommonFlt.step_7 -> G4CommonFlt.step_8 : [ after(0.3,sec) ]
    G4CommonFlt.step_8 -> G4CommonFlt.step_9 : [ after(1,sec) ]
    G4CommonFlt.step_9 -> G4CommonFlt.step_10 : [ after(6,sec) ]
    (default) -> G4CommonFlt.Run
    G4CommonFlt.Run -> G4CommonFlt.step_1
  state G4ChargeFlt
    state Run
      %% Initialize data outputs.
      AppIn_HardwiredIgn = false;
      AppIn_OBCwakeup = OBC_E.Sleep;
      AppIn_RTCwakeup = false;
      AppIn_MCUHVIL = false;
      AppIn_OBCHVIL = false;
      AppIn_SoCLEDSW = false;
      AppIn_ChgMode = Charger_Mode_E.OFF;
      AppIn_CVmodeTimer = CV_Mode_Timer_E.Off;
      AppIn_TRerror = false;
      AppIn_TRtimer = false;
      AppIn_G3CommonFlt = false;
      AppIn_G3DischargeFlt = false;
      AppIn_G4T1DischargeFlt = false;
      AppIn_G4T2DischargeFlt = false;
      AppIn_G4CommonFlt = false;
      AppIn_G4ChargeFlt = false;
      AppIn_OBCHeartbeatFail = false;
      AppIn_LoadVolt = 0;
      AppIn_PackVolt = 0;
      AppIn_ActiveDischg = Active_DisChrg_E.Inactive;
      AppIn_BattTemp = [26; 26; 26; 26; 26; 26;];
      AppIn_BattCurrent = 0;
      AppIn_BattVoltages = [4.2; 4.2; 4.2; 4.2; 4.2; 4.2; 4.2; 4.2; 4.2; 4.2; 4.2; 4.2; 4.2; 4.2; 4.2; 4.2; 4.2; 4.2; 4.2; 4.2];
      AppIn_LastStoredSOC = 0;
      AppIn_LastStoredCycle = 0;
      AppIn_I2Cerror = false;
      AppIn_LastStoredSOH = 0;
      AppIn_MachineStatus = VDU_MACHINE_STS_E.VDU_SLEEP;
      AppIn_HVMosfetfb = false;
      AppIn_DCDCMosfetfb = false;
      AppIn_PMosfetfb = false;
      AppIn_BMSVltSnsrFail = false;
      AppIn_BattPackTempSnsrFail = false;
      AppIn_VltImbFlt = false;
      AppIn_TempImbWarn = false;
      AppIn_EEPROMSoCWarn15 = false;
    state step_1
      AppIn_HardwiredIgn = true;
    state step_2
      AppIn_OBCwakeup = OBC_E.Wake_Up;
      AppIn_OBCHVIL= true;
    state step_3
      AppIn_PMosfetfb = true;
    state step_4
      AppIn_LoadVolt = 72;
      AppIn_PackVolt = 75;
    state step_5
      AppIn_HVMosfetfb = true;
    state step_6
      AppIn_DCDCMosfetfb = true;
    state step_7
      AppIn_PMosfetfb = false;
    state step_8
    state step_9
      AppIn_G4ChargeFlt = true;
    state step_10
    (default) -> G4ChargeFlt.Run
    G4ChargeFlt.Run -> G4ChargeFlt.step_1
    G4ChargeFlt.step_1 -> G4ChargeFlt.step_2 : [ after(0.2,sec) ]
    G4ChargeFlt.step_2 -> G4ChargeFlt.step_3 : [ after(0.2,sec) ]
    G4ChargeFlt.step_3 -> G4ChargeFlt.step_4 : [ after(0.3,sec) ]
    G4ChargeFlt.step_4 -> G4ChargeFlt.step_5 : [ after(0.2,sec) ]
    G4ChargeFlt.step_5 -> G4ChargeFlt.step_6 : [ after(0.3,sec) ]
    G4ChargeFlt.step_6 -> G4ChargeFlt.step_7 : [ after(0.3,sec) ]
    G4ChargeFlt.step_7 -> G4ChargeFlt.step_8 : [ after(0.3,sec) ]
    G4ChargeFlt.step_8 -> G4ChargeFlt.step_9 : [ after(1,sec) ]
    G4ChargeFlt.step_9 -> G4ChargeFlt.step_10 : [ after(6,sec) ]
  state DischgToChgIgOn
    state Run
      %% Initialize data outputs.
      AppIn_HardwiredIgn = false;
      AppIn_OBCwakeup = OBC_E.Sleep;
      AppIn_RTCwakeup = false;
      AppIn_MCUHVIL = false;
      AppIn_OBCHVIL = false;
      AppIn_SoCLEDSW = false;
      AppIn_ChgMode = Charger_Mode_E.OFF;
      AppIn_CVmodeTimer = CV_Mode_Timer_E.Off;
      AppIn_TRerror = false;
      AppIn_TRtimer = false;
      AppIn_G3CommonFlt = false;
      AppIn_G3DischargeFlt = false;
      AppIn_G4T1DischargeFlt = false;
      AppIn_G4T2DischargeFlt = false;
      AppIn_G4CommonFlt = false;
      AppIn_G4ChargeFlt = false;
      AppIn_OBCHeartbeatFail = false;
      AppIn_LoadVolt = 0;
      AppIn_PackVolt = 0;
      AppIn_ActiveDischg = Active_DisChrg_E.Inactive;
      AppIn_BattTemp = [26; 26; 26; 26; 26; 26;];
      AppIn_BattCurrent = 0;
      AppIn_BattVoltages = [4.2; 4.2; 4.2; 4.2; 4.2; 4.2; 4.2; 4.2; 4.2; 4.2; 4.2; 4.2; 4.2; 4.2; 4.2; 4.2; 4.2; 4.2; 4.2; 4.2];
      AppIn_LastStoredSOC = 0;
      AppIn_LastStoredCycle = 0;
      AppIn_I2Cerror = false;
      AppIn_LastStoredSOH = 0;
      AppIn_MachineStatus = VDU_MACHINE_STS_E.VDU_SLEEP;
      AppIn_HVMosfetfb = false;
      AppIn_DCDCMosfetfb = false;
      AppIn_PMosfetfb = false;
      AppIn_BMSVltSnsrFail = false;
      AppIn_BattPackTempSnsrFail = false;
      AppIn_VltImbFlt = false;
      AppIn_TempImbWarn = false;
      AppIn_EEPROMSoCWarn15 = false;
    state step_1
      AppIn_HardwiredIgn = true;
    state step_2
      AppIn_MCUHVIL  = true;
    state step_3
      AppIn_PMosfetfb = true;
    state step_4
      AppIn_LoadVolt = 72;
      AppIn_PackVolt = 75;
    state step_5
      AppIn_HVMosfetfb = true;
    state step_6
      AppIn_DCDCMosfetfb = true;
    state step_7
      AppIn_PMosfetfb = false;
    state step_8
    state step_9
      AppIn_OBCwakeup = OBC_E.Wake_Up;
      AppIn_OBCHVIL= true;
    state step_10
    (default) -> DischgToChgIgOn.Run
    DischgToChgIgOn.Run -> DischgToChgIgOn.step_1
    DischgToChgIgOn.step_1 -> DischgToChgIgOn.step_2 : [ after(0.2,sec) ]
    DischgToChgIgOn.step_2 -> DischgToChgIgOn.step_3 : [ after(0.2,sec) ]
    DischgToChgIgOn.step_3 -> DischgToChgIgOn.step_4 : [ after(0.3,sec) ]
    DischgToChgIgOn.step_4 -> DischgToChgIgOn.step_5 : [ after(0.2,sec) ]
    DischgToChgIgOn.step_5 -> DischgToChgIgOn.step_6 : [ after(0.3,sec) ]
    DischgToChgIgOn.step_6 -> DischgToChgIgOn.step_7 : [ after(0.3,sec) ]
    DischgToChgIgOn.step_7 -> DischgToChgIgOn.step_8 : [ after(0.3,sec) ]
    DischgToChgIgOn.step_8 -> DischgToChgIgOn.step_9 : [ after(1,sec) ]
    DischgToChgIgOn.step_9 -> DischgToChgIgOn.step_10 : [ after(0.5,sec) ]
  state FaultToSleep
    state Run
      %% Initialize data outputs.
      AppIn_HardwiredIgn = false;
      AppIn_OBCwakeup = OBC_E.Sleep;
      AppIn_RTCwakeup = false;
      AppIn_MCUHVIL = false;
      AppIn_OBCHVIL = false;
      AppIn_SoCLEDSW = false;
      AppIn_ChgMode = Charger_Mode_E.OFF;
      AppIn_CVmodeTimer = CV_Mode_Timer_E.Off;
      AppIn_TRerror = false;
      AppIn_TRtimer = false;
      AppIn_G3CommonFlt = false;
      AppIn_G3DischargeFlt = false;
      AppIn_G4T1DischargeFlt = false;
      AppIn_G4T2DischargeFlt = false;
      AppIn_G4CommonFlt = false;
      AppIn_G4ChargeFlt = false;
      AppIn_OBCHeartbeatFail = false;
      AppIn_LoadVolt = 0;
      AppIn_PackVolt = 0;
      AppIn_ActiveDischg = Active_DisChrg_E.Inactive;
      AppIn_BattTemp = [26; 26; 26; 26; 26; 26;];
      AppIn_BattCurrent = 0;
      AppIn_BattVoltages = [4.2; 4.2; 4.2; 4.2; 4.2; 4.2; 4.2; 4.2; 4.2; 4.2; 4.2; 4.2; 4.2; 4.2; 4.2; 4.2; 4.2; 4.2; 4.2; 4.2];
      AppIn_LastStoredSOC = 0;
      AppIn_LastStoredCycle = 0;
      AppIn_I2Cerror = false;
      AppIn_LastStoredSOH = 0;
      AppIn_MachineStatus = VDU_MACHINE_STS_E.VDU_SLEEP;
      AppIn_HVMosfetfb = false;
      AppIn_DCDCMosfetfb = false;
      AppIn_PMosfetfb = false;
      AppIn_BMSVltSnsrFail = false;
      AppIn_BattPackTempSnsrFail = false;
      AppIn_VltImbFlt = false;
      AppIn_TempImbWarn = false;
      AppIn_EEPROMSoCWarn15 = false;
    state step_1
      AppIn_HardwiredIgn = true;
    state step_2
      AppIn_MCUHVIL  = true;
    state step_3
      AppIn_PMosfetfb = true;
    state step_4
      AppIn_LoadVolt = 72;
      AppIn_PackVolt = 75;
    state step_5
      AppIn_HVMosfetfb = true;
    state step_6
      AppIn_DCDCMosfetfb = true;
    state step_7
      AppIn_PMosfetfb = false;
    state step_8
    state step_9
      AppIn_G4T1DischargeFlt = true;
    state step_10
      AppIn_HardwiredIgn = false;
    state step_11
    (default) -> FaultToSleep.Run
    FaultToSleep.Run -> FaultToSleep.step_1
    FaultToSleep.step_1 -> FaultToSleep.step_2 : [ after(0.2,sec) ]
    FaultToSleep.step_2 -> FaultToSleep.step_3 : [ after(0.2,sec) ]
    FaultToSleep.step_3 -> FaultToSleep.step_4 : [ after(0.3,sec) ]
    FaultToSleep.step_4 -> FaultToSleep.step_5 : [ after(0.2,sec) ]
    FaultToSleep.step_5 -> FaultToSleep.step_6 : [ after(0.3,sec) ]
    FaultToSleep.step_6 -> FaultToSleep.step_7 : [ after(0.3,sec) ]
    FaultToSleep.step_7 -> FaultToSleep.step_8 : [ after(0.3,sec) ]
    FaultToSleep.step_8 -> FaultToSleep.step_9 : [ after(1,sec) ]
    FaultToSleep.step_9 -> FaultToSleep.step_10 : [ after(6,sec) ]
    FaultToSleep.step_10 -> FaultToSleep.step_11 : [ after(11,sec) ]
  state ChgToStandbyIgOn
    state Run
      %% Initialize data outputs.
      AppIn_HardwiredIgn = false;
      AppIn_OBCwakeup = OBC_E.Sleep;
      AppIn_RTCwakeup = false;
      AppIn_MCUHVIL = false;
      AppIn_OBCHVIL = false;
      AppIn_SoCLEDSW = false;
      AppIn_ChgMode = Charger_Mode_E.OFF;
      AppIn_CVmodeTimer = CV_Mode_Timer_E.Off;
      AppIn_TRerror = false;
      AppIn_TRtimer = false;
      AppIn_G3CommonFlt = false;
      AppIn_G3DischargeFlt = false;
      AppIn_G4T1DischargeFlt = false;
      AppIn_G4T2DischargeFlt = false;
      AppIn_G4CommonFlt = false;
      AppIn_G4ChargeFlt = false;
      AppIn_OBCHeartbeatFail = false;
      AppIn_LoadVolt = 0;
      AppIn_PackVolt = 0;
      AppIn_ActiveDischg = Active_DisChrg_E.Inactive;
      AppIn_BattTemp = [26; 26; 26; 26; 26; 26;];
      AppIn_BattCurrent = 0;
      AppIn_BattVoltages = [4.2; 4.2; 4.2; 4.2; 4.2; 4.2; 4.2; 4.2; 4.2; 4.2; 4.2; 4.2; 4.2; 4.2; 4.2; 4.2; 4.2; 4.2; 4.2; 4.2];
      AppIn_LastStoredSOC = 0;
      AppIn_LastStoredCycle = 0;
      AppIn_I2Cerror = false;
      AppIn_LastStoredSOH = 0;
      AppIn_MachineStatus = VDU_MACHINE_STS_E.VDU_SLEEP;
      AppIn_HVMosfetfb = false;
      AppIn_DCDCMosfetfb = false;
      AppIn_PMosfetfb = false;
      AppIn_BMSVltSnsrFail = false;
      AppIn_BattPackTempSnsrFail = false;
      AppIn_VltImbFlt = false;
      AppIn_TempImbWarn = false;
      AppIn_EEPROMSoCWarn15 = false;
    state step_1
      AppIn_HardwiredIgn = true;
    state step_2
      AppIn_OBCwakeup = OBC_E.Wake_Up;
      AppIn_OBCHVIL= true;
    state step_3
      AppIn_PMosfetfb = true;
    state step_4
      AppIn_LoadVolt = 72;
      AppIn_PackVolt = 75;
    state step_5
      AppIn_HVMosfetfb = true;
    state step_6
      AppIn_DCDCMosfetfb = true;
    state step_7
      AppIn_PMosfetfb = false;
    state step_8
    state step_9
      AppIn_OBCwakeup = OBC_E.Sleep;
      AppIn_OBCHVIL= false;
    state step_10
      AppIn_HVMosfetfb = false;
    state step_11
    (default) -> ChgToStandbyIgOn.Run
    ChgToStandbyIgOn.Run -> ChgToStandbyIgOn.step_1
    ChgToStandbyIgOn.step_1 -> ChgToStandbyIgOn.step_2 : [ after(0.2,sec) ]
    ChgToStandbyIgOn.step_2 -> ChgToStandbyIgOn.step_3 : [ after(0.2,sec) ]
    ChgToStandbyIgOn.step_3 -> ChgToStandbyIgOn.step_4 : [ after(0.3,sec) ]
    ChgToStandbyIgOn.step_4 -> ChgToStandbyIgOn.step_5 : [ after(0.2,sec) ]
    ChgToStandbyIgOn.step_5 -> ChgToStandbyIgOn.step_6 : [ after(0.3,sec) ]
    ChgToStandbyIgOn.step_6 -> ChgToStandbyIgOn.step_7 : [ after(0.3,sec) ]
    ChgToStandbyIgOn.step_7 -> ChgToStandbyIgOn.step_8 : [ after(0.3,sec) ]
    ChgToStandbyIgOn.step_8 -> ChgToStandbyIgOn.step_9 : [ after(1,sec) ]
    ChgToStandbyIgOn.step_9 -> ChgToStandbyIgOn.step_10 : [ after(0.3,sec) ]
    ChgToStandbyIgOn.step_10 -> ChgToStandbyIgOn.step_11 : [ after(0.5,sec) ]
  state ChgToStandbyIgOff
    state Run
      %% Initialize data outputs.
      AppIn_HardwiredIgn = false;
      AppIn_OBCwakeup = OBC_E.Sleep;
      AppIn_RTCwakeup = false;
      AppIn_MCUHVIL = false;
      AppIn_OBCHVIL = false;
      AppIn_SoCLEDSW = false;
      AppIn_ChgMode = Charger_Mode_E.OFF;
      AppIn_CVmodeTimer = CV_Mode_Timer_E.Off;
      AppIn_TRerror = false;
      AppIn_TRtimer = false;
      AppIn_G3CommonFlt = false;
      AppIn_G3DischargeFlt = false;
      AppIn_G4T1DischargeFlt = false;
      AppIn_G4T2DischargeFlt = false;
      AppIn_G4CommonFlt = false;
      AppIn_G4ChargeFlt = false;
      AppIn_OBCHeartbeatFail = false;
      AppIn_LoadVolt = 0;
      AppIn_PackVolt = 0;
      AppIn_ActiveDischg = Active_DisChrg_E.Inactive;
      AppIn_BattTemp = [26; 26; 26; 26; 26; 26;];
      AppIn_BattCurrent = 0;
      AppIn_BattVoltages = [4.2; 4.2; 4.2; 4.2; 4.2; 4.2; 4.2; 4.2; 4.2; 4.2; 4.2; 4.2; 4.2; 4.2; 4.2; 4.2; 4.2; 4.2; 4.2; 4.2];
      AppIn_LastStoredSOC = 0;
      AppIn_LastStoredCycle = 0;
      AppIn_I2Cerror = false;
      AppIn_LastStoredSOH = 0;
      AppIn_MachineStatus = VDU_MACHINE_STS_E.VDU_SLEEP;
      AppIn_HVMosfetfb = false;
      AppIn_DCDCMosfetfb = false;
      AppIn_PMosfetfb = false;
      AppIn_BMSVltSnsrFail = false;
      AppIn_BattPackTempSnsrFail = false;
      AppIn_VltImbFlt = false;
      AppIn_TempImbWarn = false;
      AppIn_EEPROMSoCWarn15 = false;
    state step_1
      AppIn_OBCwakeup = OBC_E.Wake_Up;
      AppIn_OBCHVIL= true;
    state step_2
      AppIn_PMosfetfb = true;
    state step_3
      AppIn_LoadVolt = 72;
      AppIn_PackVolt = 75;
    state step_4
      AppIn_HVMosfetfb = true;
    state step_5
      AppIn_PMosfetfb = false;
    state step_6
    state step_7
      AppIn_OBCwakeup = OBC_E.Sleep;
      AppIn_OBCHVIL= false;
    state step_8
      AppIn_HVMosfetfb = false;
    state step_9
    (default) -> ChgToStandbyIgOff.Run
    ChgToStandbyIgOff.Run -> ChgToStandbyIgOff.step_1
    ChgToStandbyIgOff.step_1 -> ChgToStandbyIgOff.step_2 : [ after(0.2,sec) ]
    ChgToStandbyIgOff.step_2 -> ChgToStandbyIgOff.step_3 : [ after(0.3,sec) ]
    ChgToStandbyIgOff.step_3 -> ChgToStandbyIgOff.step_4 : [ after(0.2,sec) ]
    ChgToStandbyIgOff.step_4 -> ChgToStandbyIgOff.step_5 : [ after(0.5,sec) ]
    ChgToStandbyIgOff.step_5 -> ChgToStandbyIgOff.step_6 : [ after(0.3,sec) ]
    ChgToStandbyIgOff.step_6 -> ChgToStandbyIgOff.step_7 : [ after(1,sec) ]
    ChgToStandbyIgOff.step_7 -> ChgToStandbyIgOff.step_8 : [ after(0.3,sec) ]
    ChgToStandbyIgOff.step_8 -> ChgToStandbyIgOff.step_9 : [ after(0.5,sec) ]
  state StandbyToChargeIgOn
    state Run
      %% Initialize data outputs.
      AppIn_HardwiredIgn = false;
      AppIn_OBCwakeup = OBC_E.Sleep;
      AppIn_RTCwakeup = false;
      AppIn_MCUHVIL = false;
      AppIn_OBCHVIL = false;
      AppIn_SoCLEDSW = false;
      AppIn_ChgMode = Charger_Mode_E.OFF;
      AppIn_CVmodeTimer = CV_Mode_Timer_E.Off;
      AppIn_TRerror = false;
      AppIn_TRtimer = false;
      AppIn_G3CommonFlt = false;
      AppIn_G3DischargeFlt = false;
      AppIn_G4T1DischargeFlt = false;
      AppIn_G4T2DischargeFlt = false;
      AppIn_G4CommonFlt = false;
      AppIn_G4ChargeFlt = false;
      AppIn_OBCHeartbeatFail = false;
      AppIn_LoadVolt = 0;
      AppIn_PackVolt = 0;
      AppIn_ActiveDischg = Active_DisChrg_E.Inactive;
      AppIn_BattTemp = [26; 26; 26; 26; 26; 26;];
      AppIn_BattCurrent = 0;
      AppIn_BattVoltages = [4.2; 4.2; 4.2; 4.2; 4.2; 4.2; 4.2; 4.2; 4.2; 4.2; 4.2; 4.2; 4.2; 4.2; 4.2; 4.2; 4.2; 4.2; 4.2; 4.2];
      AppIn_LastStoredSOC = 0;
      AppIn_LastStoredCycle = 0;
      AppIn_I2Cerror = false;
      AppIn_LastStoredSOH = 0;
      AppIn_MachineStatus = VDU_MACHINE_STS_E.VDU_SLEEP;
      AppIn_HVMosfetfb = false;
      AppIn_DCDCMosfetfb = false;
      AppIn_PMosfetfb = false;
      AppIn_BMSVltSnsrFail = false;
      AppIn_BattPackTempSnsrFail = false;
      AppIn_VltImbFlt = false;
      AppIn_TempImbWarn = false;
      AppIn_EEPROMSoCWarn15 = false;
    state step_1
      AppIn_HardwiredIgn = true;
    state step_2
      AppIn_MCUHVIL  = true;
    state step_3
      AppIn_PMosfetfb = true;
    state step_4
      AppIn_LoadVolt = 72;
      AppIn_PackVolt = 75;
    state step_5
      AppIn_HVMosfetfb = true;
    state step_6
      AppIn_DCDCMosfetfb = true;
    state step_7
      AppIn_PMosfetfb = false;
    state step_8
    state step_9
      AppIn_HardwiredIgn = false;
    state step_10
      AppIn_HVMosfetfb = false;
    state step_11
      AppIn_OBCHVIL= true;
      AppIn_HardwiredIgn = true;
      AppIn_OBCwakeup = OBC_E.Wake_Up;
    state step_12
      AppIn_PMosfetfb = true;
    state step_13
      AppIn_HVMosfetfb = true;
    state step_14
      AppIn_PMosfetfb = false;
    state step_15
    (default) -> StandbyToChargeIgOn.Run
    StandbyToChargeIgOn.Run -> StandbyToChargeIgOn.step_1
    StandbyToChargeIgOn.step_1 -> StandbyToChargeIgOn.step_2 : [ after(0.2,sec) ]
    StandbyToChargeIgOn.step_2 -> StandbyToChargeIgOn.step_3 : [ after(0.2,sec) ]
    StandbyToChargeIgOn.step_3 -> StandbyToChargeIgOn.step_4 : [ after(0.3,sec) ]
    StandbyToChargeIgOn.step_4 -> StandbyToChargeIgOn.step_5 : [ after(0.2,sec) ]
    StandbyToChargeIgOn.step_5 -> StandbyToChargeIgOn.step_6 : [ after(0.3,sec) ]
    StandbyToChargeIgOn.step_6 -> StandbyToChargeIgOn.step_7 : [ after(0.3,sec) ]
    StandbyToChargeIgOn.step_7 -> StandbyToChargeIgOn.step_8 : [ after(0.3,sec) ]
    StandbyToChargeIgOn.step_8 -> StandbyToChargeIgOn.step_9 : [ after(1,sec) ]
    StandbyToChargeIgOn.step_9 -> StandbyToChargeIgOn.step_10 : [ after(0.3,sec) ]
    StandbyToChargeIgOn.step_10 -> StandbyToChargeIgOn.step_11 : [ after(0.6,sec) ]
    StandbyToChargeIgOn.step_11 -> StandbyToChargeIgOn.step_12 : [ after(0.2,sec) ]
    StandbyToChargeIgOn.step_12 -> StandbyToChargeIgOn.step_13 : [ after(0.4,sec) ]
    StandbyToChargeIgOn.step_13 -> StandbyToChargeIgOn.step_14 : [ after(0.5,sec) ]
    StandbyToChargeIgOn.step_14 -> StandbyToChargeIgOn.step_15
  state StandbyToChargeIgOff
    state Run
      %% Initialize data outputs.
      AppIn_HardwiredIgn = false;
      AppIn_OBCwakeup = OBC_E.Sleep;
      AppIn_RTCwakeup = false;
      AppIn_MCUHVIL = false;
      AppIn_OBCHVIL = false;
      AppIn_SoCLEDSW = false;
      AppIn_ChgMode = Charger_Mode_E.OFF;
      AppIn_CVmodeTimer = CV_Mode_Timer_E.Off;
      AppIn_TRerror = false;
      AppIn_TRtimer = false;
      AppIn_G3CommonFlt = false;
      AppIn_G3DischargeFlt = false;
      AppIn_G4T1DischargeFlt = false;
      AppIn_G4T2DischargeFlt = false;
      AppIn_G4CommonFlt = false;
      AppIn_G4ChargeFlt = false;
      AppIn_OBCHeartbeatFail = false;
      AppIn_LoadVolt = 0;
      AppIn_PackVolt = 0;
      AppIn_ActiveDischg = Active_DisChrg_E.Inactive;
      AppIn_BattTemp = [26; 26; 26; 26; 26; 26;];
      AppIn_BattCurrent = 0;
      AppIn_BattVoltages = [4.2; 4.2; 4.2; 4.2; 4.2; 4.2; 4.2; 4.2; 4.2; 4.2; 4.2; 4.2; 4.2; 4.2; 4.2; 4.2; 4.2; 4.2; 4.2; 4.2];
      AppIn_LastStoredSOC = 0;
      AppIn_LastStoredCycle = 0;
      AppIn_I2Cerror = false;
      AppIn_LastStoredSOH = 0;
      AppIn_MachineStatus = VDU_MACHINE_STS_E.VDU_SLEEP;
      AppIn_HVMosfetfb = false;
      AppIn_DCDCMosfetfb = false;
      AppIn_PMosfetfb = false;
      AppIn_BMSVltSnsrFail = false;
      AppIn_BattPackTempSnsrFail = false;
      AppIn_VltImbFlt = false;
      AppIn_TempImbWarn = false;
      AppIn_EEPROMSoCWarn15 = false;
    state step_1
      AppIn_HardwiredIgn = true;
    state step_2
      AppIn_MCUHVIL  = true;
    state step_3
      AppIn_PMosfetfb = true;
    state step_4
      AppIn_LoadVolt = 72;
      AppIn_PackVolt = 75;
    state step_5
      AppIn_HVMosfetfb = true;
    state step_6
      AppIn_DCDCMosfetfb = true;
    state step_7
      AppIn_PMosfetfb = false;
    state step_8
    state step_9
      AppIn_HardwiredIgn = false;
    state step_10
      AppIn_HVMosfetfb = false;
    state step_11
      AppIn_OBCwakeup = OBC_E.Wake_Up;
      AppIn_OBCHVIL= true;
    state step_12
      AppIn_PMosfetfb = true;
    state step_13
      AppIn_HVMosfetfb = true;
    state step_14
      AppIn_DCDCMosfetfb = false;
    state step_15
      AppIn_PMosfetfb = false;
    state step_16
    (default) -> StandbyToChargeIgOff.Run
    StandbyToChargeIgOff.Run -> StandbyToChargeIgOff.step_1
    StandbyToChargeIgOff.step_1 -> StandbyToChargeIgOff.step_2 : [ after(0.2,sec) ]
    StandbyToChargeIgOff.step_2 -> StandbyToChargeIgOff.step_3 : [ after(0.2,sec) ]
    StandbyToChargeIgOff.step_3 -> StandbyToChargeIgOff.step_4 : [ after(0.3,sec) ]
    StandbyToChargeIgOff.step_4 -> StandbyToChargeIgOff.step_5 : [ after(0.2,sec) ]
    StandbyToChargeIgOff.step_5 -> StandbyToChargeIgOff.step_6 : [ after(0.3,sec) ]
    StandbyToChargeIgOff.step_6 -> StandbyToChargeIgOff.step_7 : [ after(0.3,sec) ]
    StandbyToChargeIgOff.step_7 -> StandbyToChargeIgOff.step_8 : [ after(0.3,sec) ]
    StandbyToChargeIgOff.step_8 -> StandbyToChargeIgOff.step_9 : [ after(1,sec) ]
    StandbyToChargeIgOff.step_9 -> StandbyToChargeIgOff.step_10 : [ after(0.3,sec) ]
    StandbyToChargeIgOff.step_10 -> StandbyToChargeIgOff.step_11 : [ after(0.6,sec) ]
    StandbyToChargeIgOff.step_11 -> StandbyToChargeIgOff.step_12 : [ after(0.2,sec) ]
    StandbyToChargeIgOff.step_12 -> StandbyToChargeIgOff.step_13 : [ after(0.4,sec) ]
    StandbyToChargeIgOff.step_13 -> StandbyToChargeIgOff.step_14 : [ after(0.3,sec) ]
    StandbyToChargeIgOff.step_14 -> StandbyToChargeIgOff.step_15 : [ after(0.3,sec) ]
    StandbyToChargeIgOff.step_15 -> StandbyToChargeIgOff.step_16 : [ after(1,sec) ]
  state ChgToFltIgOff
    state Run
      %% Initialize data outputs.
      AppIn_HardwiredIgn = false;
      AppIn_OBCwakeup = OBC_E.Sleep;
      AppIn_RTCwakeup = false;
      AppIn_MCUHVIL = false;
      AppIn_OBCHVIL = false;
      AppIn_SoCLEDSW = false;
      AppIn_ChgMode = Charger_Mode_E.OFF;
      AppIn_CVmodeTimer = CV_Mode_Timer_E.Off;
      AppIn_TRerror = false;
      AppIn_TRtimer = false;
      AppIn_G3CommonFlt = false;
      AppIn_G3DischargeFlt = false;
      AppIn_G4T1DischargeFlt = false;
      AppIn_G4T2DischargeFlt = false;
      AppIn_G4CommonFlt = false;
      AppIn_G4ChargeFlt = false;
      AppIn_OBCHeartbeatFail = false;
      AppIn_LoadVolt = 0;
      AppIn_PackVolt = 0;
      AppIn_ActiveDischg = Active_DisChrg_E.Inactive;
      AppIn_BattTemp = [26; 26; 26; 26; 26; 26;];
      AppIn_BattCurrent = 0;
      AppIn_BattVoltages = [4.2; 4.2; 4.2; 4.2; 4.2; 4.2; 4.2; 4.2; 4.2; 4.2; 4.2; 4.2; 4.2; 4.2; 4.2; 4.2; 4.2; 4.2; 4.2; 4.2];
      AppIn_LastStoredSOC = 0;
      AppIn_LastStoredCycle = 0;
      AppIn_I2Cerror = false;
      AppIn_LastStoredSOH = 0;
      AppIn_MachineStatus = VDU_MACHINE_STS_E.VDU_SLEEP;
      AppIn_HVMosfetfb = false;
      AppIn_DCDCMosfetfb = false;
      AppIn_PMosfetfb = false;
      AppIn_BMSVltSnsrFail = false;
      AppIn_BattPackTempSnsrFail = false;
      AppIn_VltImbFlt = false;
      AppIn_TempImbWarn = false;
      AppIn_EEPROMSoCWarn15 = false;
    state step_1
      AppIn_OBCwakeup = OBC_E.Wake_Up;
      AppIn_OBCHVIL= true;
    state step_2
      AppIn_PMosfetfb = true;
    state step_3
      AppIn_LoadVolt = 72;
      AppIn_PackVolt = 75;
    state step_4
      AppIn_HVMosfetfb = true;
    state step_5
      AppIn_PMosfetfb = false;
    state step_6
    state step_7
      AppIn_G4ChargeFlt = true;
    state step_8
      AppIn_OBCwakeup = OBC_E.Sleep;
    (default) -> ChgToFltIgOff.Run
    ChgToFltIgOff.Run -> ChgToFltIgOff.step_1
    ChgToFltIgOff.step_1 -> ChgToFltIgOff.step_2 : [ after(0.2,sec) ]
    ChgToFltIgOff.step_2 -> ChgToFltIgOff.step_3 : [ after(0.3,sec) ]
    ChgToFltIgOff.step_3 -> ChgToFltIgOff.step_4 : [ after(0.2,sec) ]
    ChgToFltIgOff.step_4 -> ChgToFltIgOff.step_5 : [ after(0.5,sec) ]
    ChgToFltIgOff.step_5 -> ChgToFltIgOff.step_6 : [ after(0.3,sec) ]
    ChgToFltIgOff.step_6 -> ChgToFltIgOff.step_7 : [ after(1,sec) ]
    ChgToFltIgOff.step_7 -> ChgToFltIgOff.step_8 : [ after(6,sec) ]
  state FltToChgIgOff
    state Run
      %% Initialize data outputs.
      AppIn_HardwiredIgn = false;
      AppIn_OBCwakeup = OBC_E.Sleep;
      AppIn_RTCwakeup = false;
      AppIn_MCUHVIL = false;
      AppIn_OBCHVIL = false;
      AppIn_SoCLEDSW = false;
      AppIn_ChgMode = Charger_Mode_E.OFF;
      AppIn_CVmodeTimer = CV_Mode_Timer_E.Off;
      AppIn_TRerror = false;
      AppIn_TRtimer = false;
      AppIn_G3CommonFlt = false;
      AppIn_G3DischargeFlt = false;
      AppIn_G4T1DischargeFlt = false;
      AppIn_G4T2DischargeFlt = false;
      AppIn_G4CommonFlt = false;
      AppIn_G4ChargeFlt = false;
      AppIn_OBCHeartbeatFail = false;
      AppIn_LoadVolt = 0;
      AppIn_PackVolt = 0;
      AppIn_ActiveDischg = Active_DisChrg_E.Inactive;
      AppIn_BattTemp = [26; 26; 26; 26; 26; 26;];
      AppIn_BattCurrent = 0;
      AppIn_BattVoltages = [4.2; 4.2; 4.2; 4.2; 4.2; 4.2; 4.2; 4.2; 4.2; 4.2; 4.2; 4.2; 4.2; 4.2; 4.2; 4.2; 4.2; 4.2; 4.2; 4.2];
      AppIn_LastStoredSOC = 0;
      AppIn_LastStoredCycle = 0;
      AppIn_I2Cerror = false;
      AppIn_LastStoredSOH = 0;
      AppIn_MachineStatus = VDU_MACHINE_STS_E.VDU_SLEEP;
      AppIn_HVMosfetfb = false;
      AppIn_DCDCMosfetfb = false;
      AppIn_PMosfetfb = false;
      AppIn_BMSVltSnsrFail = false;
      AppIn_BattPackTempSnsrFail = false;
      AppIn_VltImbFlt = false;
      AppIn_TempImbWarn = false;
      AppIn_EEPROMSoCWarn15 = false;
    state step_1
      AppIn_HardwiredIgn = true;
    state step_2
      AppIn_MCUHVIL  = true;
    state step_3
      AppIn_PMosfetfb = true;
    state step_4
      AppIn_LoadVolt = 72;
      AppIn_PackVolt = 75;
    state step_5
      AppIn_HVMosfetfb = true;
    state step_6
      AppIn_DCDCMosfetfb = true;
    state step_7
      AppIn_PMosfetfb = false;
    state step_8
    state step_9
      AppIn_G4T2DischargeFlt = true;
    state step_10
      AppIn_HardwiredIgn = false;
    state step_11
      AppIn_G4T2DischargeFlt = false;
      AppIn_OBCwakeup = OBC_E.Wake_Up;
      AppIn_OBCHVIL= true;
    state step_12
      AppIn_PMosfetfb = true;
    state step_13
      AppIn_HVMosfetfb = true;
    state step_14
      AppIn_DCDCMosfetfb = false;
    state step_15
      AppIn_PMosfetfb = false;
    state step_16
    (default) -> FltToChgIgOff.Run
    FltToChgIgOff.Run -> FltToChgIgOff.step_1
    FltToChgIgOff.step_1 -> FltToChgIgOff.step_2 : [ after(0.2,sec) ]
    FltToChgIgOff.step_2 -> FltToChgIgOff.step_3 : [ after(0.2,sec) ]
    FltToChgIgOff.step_3 -> FltToChgIgOff.step_4 : [ after(0.3,sec) ]
    FltToChgIgOff.step_4 -> FltToChgIgOff.step_5 : [ after(0.2,sec) ]
    FltToChgIgOff.step_5 -> FltToChgIgOff.step_6 : [ after(0.3,sec) ]
    FltToChgIgOff.step_6 -> FltToChgIgOff.step_7 : [ after(0.3,sec) ]
    FltToChgIgOff.step_7 -> FltToChgIgOff.step_8 : [ after(0.3,sec) ]
    FltToChgIgOff.step_8 -> FltToChgIgOff.step_9 : [ after(1,sec) ]
    FltToChgIgOff.step_9 -> FltToChgIgOff.step_10 : [ after(6,sec) ]
    FltToChgIgOff.step_10 -> FltToChgIgOff.step_11 : [ after(0.2,sec) ]
    FltToChgIgOff.step_11 -> FltToChgIgOff.step_12 : [ after(0.2,sec) ]
    FltToChgIgOff.step_12 -> FltToChgIgOff.step_13 : [ after(0.4,sec) ]
    FltToChgIgOff.step_13 -> FltToChgIgOff.step_14 : [ after(0.3,sec) ]
    FltToChgIgOff.step_14 -> FltToChgIgOff.step_15 : [ after(0.3,sec) ]
    FltToChgIgOff.step_15 -> FltToChgIgOff.step_16 : [ after(1,sec) ]
  state FltToChgIgOn
    state Run
      %% Initialize data outputs.
      AppIn_HardwiredIgn = false;
      AppIn_OBCwakeup = OBC_E.Sleep;
      AppIn_RTCwakeup = false;
      AppIn_MCUHVIL = false;
      AppIn_OBCHVIL = false;
      AppIn_SoCLEDSW = false;
      AppIn_ChgMode = Charger_Mode_E.OFF;
      AppIn_CVmodeTimer = CV_Mode_Timer_E.Off;
      AppIn_TRerror = false;
      AppIn_TRtimer = false;
      AppIn_G3CommonFlt = false;
      AppIn_G3DischargeFlt = false;
      AppIn_G4T1DischargeFlt = false;
      AppIn_G4T2DischargeFlt = false;
      AppIn_G4CommonFlt = false;
      AppIn_G4ChargeFlt = false;
      AppIn_OBCHeartbeatFail = false;
      AppIn_LoadVolt = 0;
      AppIn_PackVolt = 0;
      AppIn_ActiveDischg = Active_DisChrg_E.Inactive;
      AppIn_BattTemp = [26; 26; 26; 26; 26; 26;];
      AppIn_BattCurrent = 0;
      AppIn_BattVoltages = [4.2; 4.2; 4.2; 4.2; 4.2; 4.2; 4.2; 4.2; 4.2; 4.2; 4.2; 4.2; 4.2; 4.2; 4.2; 4.2; 4.2; 4.2; 4.2; 4.2];
      AppIn_LastStoredSOC = 0;
      AppIn_LastStoredCycle = 0;
      AppIn_I2Cerror = false;
      AppIn_LastStoredSOH = 0;
      AppIn_MachineStatus = VDU_MACHINE_STS_E.VDU_SLEEP;
      AppIn_HVMosfetfb = false;
      AppIn_DCDCMosfetfb = false;
      AppIn_PMosfetfb = false;
      AppIn_BMSVltSnsrFail = false;
      AppIn_BattPackTempSnsrFail = false;
      AppIn_VltImbFlt = false;
      AppIn_TempImbWarn = false;
      AppIn_EEPROMSoCWarn15 = false;
    state step_1
      AppIn_HardwiredIgn = true;
    state step_2
      AppIn_MCUHVIL  = true;
    state step_3
      AppIn_PMosfetfb = true;
    state step_4
      AppIn_LoadVolt = 72;
      AppIn_PackVolt = 75;
    state step_5
      AppIn_HVMosfetfb = true;
    state step_6
      AppIn_DCDCMosfetfb = true;
    state step_7
      AppIn_PMosfetfb = false;
    state step_8
    state step_9
      AppIn_G4T1DischargeFlt = true;
    state step_10
    state step_11
      AppIn_G4T1DischargeFlt = false;
      AppIn_HardwiredIgn = true;
      AppIn_OBCwakeup = OBC_E.Wake_Up;
      AppIn_OBCHVIL= true;
    state step_12
      AppIn_PMosfetfb = true;
    state step_13
      AppIn_HVMosfetfb = true;
    state step_14
      AppIn_PMosfetfb = false;
    state step_15
    (default) -> FltToChgIgOn.Run
    FltToChgIgOn.Run -> FltToChgIgOn.step_1
    FltToChgIgOn.step_1 -> FltToChgIgOn.step_2 : [ after(0.2,sec) ]
    FltToChgIgOn.step_2 -> FltToChgIgOn.step_3 : [ after(0.2,sec) ]
    FltToChgIgOn.step_3 -> FltToChgIgOn.step_4 : [ after(0.3,sec) ]
    FltToChgIgOn.step_4 -> FltToChgIgOn.step_5 : [ after(0.2,sec) ]
    FltToChgIgOn.step_5 -> FltToChgIgOn.step_6 : [ after(0.3,sec) ]
    FltToChgIgOn.step_6 -> FltToChgIgOn.step_7 : [ after(0.3,sec) ]
    FltToChgIgOn.step_7 -> FltToChgIgOn.step_8 : [ after(0.3,sec) ]
    FltToChgIgOn.step_8 -> FltToChgIgOn.step_9 : [ after(1,sec) ]
    FltToChgIgOn.step_9 -> FltToChgIgOn.step_10 : [ after(6,sec) ]
    FltToChgIgOn.step_10 -> FltToChgIgOn.step_11 : [ after(0.2,sec) ]
    FltToChgIgOn.step_11 -> FltToChgIgOn.step_12 : [ after(0.2,sec) ]
    FltToChgIgOn.step_12 -> FltToChgIgOn.step_13 : [ after(0.4,sec) ]
    FltToChgIgOn.step_13 -> FltToChgIgOn.step_14 : [ after(0.5,sec) ]
    FltToChgIgOn.step_14 -> FltToChgIgOn.step_15 : [ after(1,sec) ]
  state PrechgVoltFltWhenIgOn
    state Run
      %% Initialize data outputs.
      AppIn_HardwiredIgn = false;
      AppIn_OBCwakeup = OBC_E.Sleep;
      AppIn_RTCwakeup = false;
      AppIn_MCUHVIL = false;
      AppIn_OBCHVIL = false;
      AppIn_SoCLEDSW = false;
      AppIn_ChgMode = Charger_Mode_E.OFF;
      AppIn_CVmodeTimer = CV_Mode_Timer_E.Off;
      AppIn_TRerror = false;
      AppIn_TRtimer = false;
      AppIn_G3CommonFlt = false;
      AppIn_G3DischargeFlt = false;
      AppIn_G4T1DischargeFlt = false;
      AppIn_G4T2DischargeFlt = false;
      AppIn_G4CommonFlt = false;
      AppIn_G4ChargeFlt = false;
      AppIn_OBCHeartbeatFail = false;
      AppIn_LoadVolt = 0;
      AppIn_PackVolt = 0;
      AppIn_ActiveDischg = Active_DisChrg_E.Inactive;
      AppIn_BattTemp = [26; 26; 26; 26; 26; 26;];
      AppIn_BattCurrent = 0;
      AppIn_BattVoltages = [4.2; 4.2; 4.2; 4.2; 4.2; 4.2; 4.2; 4.2; 4.2; 4.2; 4.2; 4.2; 4.2; 4.2; 4.2; 4.2; 4.2; 4.2; 4.2; 4.2];
      AppIn_LastStoredSOC = 0;
      AppIn_LastStoredCycle = 0;
      AppIn_I2Cerror = false;
      AppIn_LastStoredSOH = 0;
      AppIn_MachineStatus = VDU_MACHINE_STS_E.VDU_SLEEP;
      AppIn_HVMosfetfb = false;
      AppIn_DCDCMosfetfb = false;
      AppIn_PMosfetfb = false;
      AppIn_BMSVltSnsrFail = false;
      AppIn_BattPackTempSnsrFail = false;
      AppIn_VltImbFlt = false;
      AppIn_TempImbWarn = false;
      AppIn_EEPROMSoCWarn15 = false;
    state step_1
      AppIn_HardwiredIgn = true;
    state step_2
      AppIn_MCUHVIL = true;
    state step_3
      AppIn_PMosfetfb = true;
    state step_4
      AppIn_LoadVolt = 55;
      AppIn_PackVolt = 60;
    state step_5
    state step_6
      AppIn_G4CommonFlt = true;
    (default) -> PrechgVoltFltWhenIgOn.Run
    PrechgVoltFltWhenIgOn.Run -> PrechgVoltFltWhenIgOn.step_1
    PrechgVoltFltWhenIgOn.step_1 -> PrechgVoltFltWhenIgOn.step_2 : [ after(0.1,sec) ]
    PrechgVoltFltWhenIgOn.step_2 -> PrechgVoltFltWhenIgOn.step_3 : [ after(0.1,sec) ]
    PrechgVoltFltWhenIgOn.step_3 -> PrechgVoltFltWhenIgOn.step_4 : [ after(0.2,sec) ]
    PrechgVoltFltWhenIgOn.step_4 -> PrechgVoltFltWhenIgOn.step_5 : [ after(0.5,sec) ]
    PrechgVoltFltWhenIgOn.step_5 -> PrechgVoltFltWhenIgOn.step_6 : [ after(0.1,sec) ]
  state PrechgVoltFltWhenIgOff
    state Run
      %% Initialize data outputs.
      AppIn_HardwiredIgn = false;
      AppIn_OBCwakeup = OBC_E.Sleep;
      AppIn_RTCwakeup = false;
      AppIn_MCUHVIL = false;
      AppIn_OBCHVIL = false;
      AppIn_SoCLEDSW = false;
      AppIn_ChgMode = Charger_Mode_E.OFF;
      AppIn_CVmodeTimer = CV_Mode_Timer_E.Off;
      AppIn_TRerror = false;
      AppIn_TRtimer = false;
      AppIn_G3CommonFlt = false;
      AppIn_G3DischargeFlt = false;
      AppIn_G4T1DischargeFlt = false;
      AppIn_G4T2DischargeFlt = false;
      AppIn_G4CommonFlt = false;
      AppIn_G4ChargeFlt = false;
      AppIn_OBCHeartbeatFail = false;
      AppIn_LoadVolt = 0;
      AppIn_PackVolt = 0;
      AppIn_ActiveDischg = Active_DisChrg_E.Inactive;
      AppIn_BattTemp = [26; 26; 26; 26; 26; 26;];
      AppIn_BattCurrent = 0;
      AppIn_BattVoltages = [4.2; 4.2; 4.2; 4.2; 4.2; 4.2; 4.2; 4.2; 4.2; 4.2; 4.2; 4.2; 4.2; 4.2; 4.2; 4.2; 4.2; 4.2; 4.2; 4.2];
      AppIn_LastStoredSOC = 0;
      AppIn_LastStoredCycle = 0;
      AppIn_I2Cerror = false;
      AppIn_LastStoredSOH = 0;
      AppIn_MachineStatus = VDU_MACHINE_STS_E.VDU_SLEEP;
      AppIn_HVMosfetfb = false;
      AppIn_DCDCMosfetfb = false;
      AppIn_PMosfetfb = false;
      AppIn_BMSVltSnsrFail = false;
      AppIn_BattPackTempSnsrFail = false;
      AppIn_VltImbFlt = false;
      AppIn_TempImbWarn = false;
      AppIn_EEPROMSoCWarn15 = false;
    state step_1
      AppIn_OBCwakeup = OBC_E.Wake_Up;
      AppIn_OBCHVIL = true;
    state step_2
      AppIn_PMosfetfb = true;
    state step_3
      AppIn_LoadVolt = 55;
      AppIn_PackVolt = 60;
    state step_4
    state step_5
      AppIn_G4CommonFlt = true;
      AppIn_HardwiredIgn = true;
    (default) -> PrechgVoltFltWhenIgOff.Run
    PrechgVoltFltWhenIgOff.Run -> PrechgVoltFltWhenIgOff.step_1
    PrechgVoltFltWhenIgOff.step_1 -> PrechgVoltFltWhenIgOff.step_2 : [ after(0.2,sec) ]
    PrechgVoltFltWhenIgOff.step_2 -> PrechgVoltFltWhenIgOff.step_3 : [ after(0.2,sec) ]
    PrechgVoltFltWhenIgOff.step_3 -> PrechgVoltFltWhenIgOff.step_4 : [ after(0.5,sec) ]
    PrechgVoltFltWhenIgOff.step_4 -> PrechgVoltFltWhenIgOff.step_5 : [ after(0.1,sec) ]
  state ChargeSequenceIgOff
    state Run
      %% Initialize data outputs.
      AppIn_HardwiredIgn = false;
      AppIn_OBCwakeup = OBC_E.Sleep;
      AppIn_RTCwakeup = false;
      AppIn_MCUHVIL = false;
      AppIn_OBCHVIL = false;
      AppIn_SoCLEDSW = false;
      AppIn_ChgMode = Charger_Mode_E.OFF;
      AppIn_CVmodeTimer = CV_Mode_Timer_E.Off;
      AppIn_TRerror = false;
      AppIn_TRtimer = false;
      AppIn_G3CommonFlt = false;
      AppIn_G3DischargeFlt = false;
      AppIn_G4T1DischargeFlt = false;
      AppIn_G4T2DischargeFlt = false;
      AppIn_G4CommonFlt = false;
      AppIn_G4ChargeFlt = false;
      AppIn_OBCHeartbeatFail = false;
      AppIn_LoadVolt = 0;
      AppIn_PackVolt = 0;
      AppIn_ActiveDischg = Active_DisChrg_E.Inactive;
      AppIn_BattTemp = [26; 26; 26; 26; 26; 26;];
      AppIn_BattCurrent = 0;
      AppIn_BattVoltages = [4.2; 4.2; 4.2; 4.2; 4.2; 4.2; 4.2; 4.2; 4.2; 4.2; 4.2; 4.2; 4.2; 4.2; 4.2; 4.2; 4.2; 4.2; 4.2; 4.2];
      AppIn_LastStoredSOC = 0;
      AppIn_LastStoredCycle = 0;
      AppIn_I2Cerror = false;
      AppIn_LastStoredSOH = 0;
      AppIn_MachineStatus = VDU_MACHINE_STS_E.VDU_SLEEP;
      AppIn_HVMosfetfb = false;
      AppIn_DCDCMosfetfb = false;
      AppIn_PMosfetfb = false;
      AppIn_BMSVltSnsrFail = false;
      AppIn_BattPackTempSnsrFail = false;
      AppIn_VltImbFlt = false;
      AppIn_TempImbWarn = false;
      AppIn_EEPROMSoCWarn15 = false;
    state step_1
      AppIn_OBCwakeup = OBC_E.Wake_Up;
      AppIn_OBCHVIL= true;
    state step_2
      AppIn_PMosfetfb = true;
    state step_3
      AppIn_LoadVolt = 72;
      AppIn_PackVolt = 75;
    state step_4
      AppIn_HVMosfetfb = true;
    state step_5
      AppIn_PMosfetfb = false;
    state step_6
    state step_7
      AppIn_HardwiredIgn = true;
    state step_8
      AppIn_HardwiredIgn = false;
    (default) -> ChargeSequenceIgOff.Run
    ChargeSequenceIgOff.Run -> ChargeSequenceIgOff.step_1
    ChargeSequenceIgOff.step_1 -> ChargeSequenceIgOff.step_2 : [ after(0.2,sec) ]
    ChargeSequenceIgOff.step_2 -> ChargeSequenceIgOff.step_3 : [ after(0.3,sec) ]
    ChargeSequenceIgOff.step_3 -> ChargeSequenceIgOff.step_4 : [ after(0.2,sec) ]
    ChargeSequenceIgOff.step_4 -> ChargeSequenceIgOff.step_5 : [ after(0.5,sec) ]
    ChargeSequenceIgOff.step_5 -> ChargeSequenceIgOff.step_6 : [ after(0.3,sec) ]
    ChargeSequenceIgOff.step_6 -> ChargeSequenceIgOff.step_7 : [ after(1,sec) ]
    ChargeSequenceIgOff.step_7 -> ChargeSequenceIgOff.step_8 : [ after(0.2,sec) ]
  state ChargeSequenceIgOn
    state Run
      %% Initialize data outputs.
      AppIn_HardwiredIgn = false;
      AppIn_OBCwakeup = OBC_E.Sleep;
      AppIn_RTCwakeup = false;
      AppIn_MCUHVIL = false;
      AppIn_OBCHVIL = false;
      AppIn_SoCLEDSW = false;
      AppIn_ChgMode = Charger_Mode_E.OFF;
      AppIn_CVmodeTimer = CV_Mode_Timer_E.Off;
      AppIn_TRerror = false;
      AppIn_TRtimer = false;
      AppIn_G3CommonFlt = false;
      AppIn_G3DischargeFlt = false;
      AppIn_G4T1DischargeFlt = false;
      AppIn_G4T2DischargeFlt = false;
      AppIn_G4CommonFlt = false;
      AppIn_G4ChargeFlt = false;
      AppIn_OBCHeartbeatFail = false;
      AppIn_LoadVolt = 0;
      AppIn_PackVolt = 0;
      AppIn_ActiveDischg = Active_DisChrg_E.Inactive;
      AppIn_BattTemp = [26; 26; 26; 26; 26; 26;];
      AppIn_BattCurrent = 0;
      AppIn_BattVoltages = [4.2; 4.2; 4.2; 4.2; 4.2; 4.2; 4.2; 4.2; 4.2; 4.2; 4.2; 4.2; 4.2; 4.2; 4.2; 4.2; 4.2; 4.2; 4.2; 4.2];
      AppIn_LastStoredSOC = 0;
      AppIn_LastStoredCycle = 0;
      AppIn_I2Cerror = false;
      AppIn_LastStoredSOH = 0;
      AppIn_MachineStatus = VDU_MACHINE_STS_E.VDU_SLEEP;
      AppIn_HVMosfetfb = false;
      AppIn_DCDCMosfetfb = false;
      AppIn_PMosfetfb = false;
      AppIn_BMSVltSnsrFail = false;
      AppIn_BattPackTempSnsrFail = false;
      AppIn_VltImbFlt = false;
      AppIn_TempImbWarn = false;
      AppIn_EEPROMSoCWarn15 = false;
    state step_1
      AppIn_HardwiredIgn = true;
    state step_2
      AppIn_OBCwakeup = OBC_E.Wake_Up;
      AppIn_OBCHVIL= true;
    state step_3
      AppIn_PMosfetfb = true;
    state step_4
      AppIn_LoadVolt = 72;
      AppIn_PackVolt = 75;
    state step_5
      AppIn_HVMosfetfb = true;
    state step_6
      AppIn_DCDCMosfetfb = true;
    state step_7
      AppIn_PMosfetfb = false;
    state step_8
    state step_9
      AppIn_HardwiredIgn = false;
      AppIn_ActiveDischg = Active_DisChrg_E.Completed;
    state step_10
      AppIn_HardwiredIgn = true;
    (default) -> ChargeSequenceIgOn.Run
    ChargeSequenceIgOn.Run -> ChargeSequenceIgOn.step_1
    ChargeSequenceIgOn.step_1 -> ChargeSequenceIgOn.step_2 : [ after(0.2,sec) ]
    ChargeSequenceIgOn.step_2 -> ChargeSequenceIgOn.step_3 : [ after(0.2,sec) ]
    ChargeSequenceIgOn.step_3 -> ChargeSequenceIgOn.step_4 : [ after(0.3,sec) ]
    ChargeSequenceIgOn.step_4 -> ChargeSequenceIgOn.step_5 : [ after(0.2,sec) ]
    ChargeSequenceIgOn.step_5 -> ChargeSequenceIgOn.step_6 : [ after(0.3,sec) ]
    ChargeSequenceIgOn.step_6 -> ChargeSequenceIgOn.step_7 : [ after(0.3,sec) ]
    ChargeSequenceIgOn.step_7 -> ChargeSequenceIgOn.step_8 : [ after(0.3,sec) ]
    ChargeSequenceIgOn.step_8 -> ChargeSequenceIgOn.step_9 : [ after(1,sec) ]
    ChargeSequenceIgOn.step_9 -> ChargeSequenceIgOn.step_10 : [ after(0.3,sec) ]
  state DischgToChargeAndIgOnToOff
    state Run
      %% Initialize data outputs.
      AppIn_HardwiredIgn = false;
      AppIn_OBCwakeup = OBC_E.Sleep;
      AppIn_RTCwakeup = false;
      AppIn_MCUHVIL = false;
      AppIn_OBCHVIL = false;
      AppIn_SoCLEDSW = false;
      AppIn_ChgMode = Charger_Mode_E.OFF;
      AppIn_CVmodeTimer = CV_Mode_Timer_E.Off;
      AppIn_TRerror = false;
      AppIn_TRtimer = false;
      AppIn_G3CommonFlt = false;
      AppIn_G3DischargeFlt = false;
      AppIn_G4T1DischargeFlt = false;
      AppIn_G4T2DischargeFlt = false;
      AppIn_G4CommonFlt = false;
      AppIn_G4ChargeFlt = false;
      AppIn_OBCHeartbeatFail = false;
      AppIn_LoadVolt = 0;
      AppIn_PackVolt = 0;
      AppIn_ActiveDischg = Active_DisChrg_E.Inactive;
      AppIn_BattTemp = [26; 26; 26; 26; 26; 26;];
      AppIn_BattCurrent = 0;
      AppIn_BattVoltages = [4.2; 4.2; 4.2; 4.2; 4.2; 4.2; 4.2; 4.2; 4.2; 4.2; 4.2; 4.2; 4.2; 4.2; 4.2; 4.2; 4.2; 4.2; 4.2; 4.2];
      AppIn_LastStoredSOC = 0;
      AppIn_LastStoredCycle = 0;
      AppIn_I2Cerror = false;
      AppIn_LastStoredSOH = 0;
      AppIn_MachineStatus = VDU_MACHINE_STS_E.VDU_SLEEP;
      AppIn_HVMosfetfb = false;
      AppIn_DCDCMosfetfb = false;
      AppIn_PMosfetfb = false;
      AppIn_BMSVltSnsrFail = false;
      AppIn_BattPackTempSnsrFail = false;
      AppIn_VltImbFlt = false;
      AppIn_TempImbWarn = false;
      AppIn_EEPROMSoCWarn15 = false;
    state step_1
      AppIn_HardwiredIgn = true;
    state step_2
      AppIn_MCUHVIL  = true;
    state step_3
      AppIn_PMosfetfb = true;
    state step_4
      AppIn_LoadVolt = 72;
      AppIn_PackVolt = 75;
    state step_5
      AppIn_HVMosfetfb = true;
    state step_6
      AppIn_DCDCMosfetfb = true;
    state step_7
      AppIn_PMosfetfb = false;
    state step_8
    state step_9
      AppIn_OBCwakeup = OBC_E.Wake_Up;
      AppIn_OBCHVIL= true;
    state step_10
    state step_11
      AppIn_HardwiredIgn = false;
    (default) -> DischgToChargeAndIgOnToOff.Run
    DischgToChargeAndIgOnToOff.Run -> DischgToChargeAndIgOnToOff.step_1
    DischgToChargeAndIgOnToOff.step_1 -> DischgToChargeAndIgOnToOff.step_2 : [ after(0.2,sec) ]
    DischgToChargeAndIgOnToOff.step_2 -> DischgToChargeAndIgOnToOff.step_3 : [ after(0.2,sec) ]
    DischgToChargeAndIgOnToOff.step_3 -> DischgToChargeAndIgOnToOff.step_4 : [ after(0.3,sec) ]
    DischgToChargeAndIgOnToOff.step_4 -> DischgToChargeAndIgOnToOff.step_5 : [ after(0.2,sec) ]
    DischgToChargeAndIgOnToOff.step_5 -> DischgToChargeAndIgOnToOff.step_6 : [ after(0.3,sec) ]
    DischgToChargeAndIgOnToOff.step_6 -> DischgToChargeAndIgOnToOff.step_7 : [ after(0.3,sec) ]
    DischgToChargeAndIgOnToOff.step_7 -> DischgToChargeAndIgOnToOff.step_8 : [ after(0.3,sec) ]
    DischgToChargeAndIgOnToOff.step_8 -> DischgToChargeAndIgOnToOff.step_9 : [ after(1,sec) ]
    DischgToChargeAndIgOnToOff.step_9 -> DischgToChargeAndIgOnToOff.step_10 : [ after(0.5,sec) ]
    DischgToChargeAndIgOnToOff.step_10 -> DischgToChargeAndIgOnToOff.step_11 : [ after(1,sec) ]
  state G4T2DischargeToSleep
    state Run
      %% Initialize data outputs.
      AppIn_HardwiredIgn = false;
      AppIn_OBCwakeup = OBC_E.Sleep;
      AppIn_RTCwakeup = false;
      AppIn_MCUHVIL = false;
      AppIn_OBCHVIL = false;
      AppIn_SoCLEDSW = false;
      AppIn_ChgMode = Charger_Mode_E.OFF;
      AppIn_CVmodeTimer = CV_Mode_Timer_E.Off;
      AppIn_TRerror = false;
      AppIn_TRtimer = false;
      AppIn_G3CommonFlt = false;
      AppIn_G3DischargeFlt = false;
      AppIn_G4T1DischargeFlt = false;
      AppIn_G4T2DischargeFlt = false;
      AppIn_G4CommonFlt = false;
      AppIn_G4ChargeFlt = false;
      AppIn_OBCHeartbeatFail = false;
      AppIn_LoadVolt = 0;
      AppIn_PackVolt = 0;
      AppIn_ActiveDischg = Active_DisChrg_E.Inactive;
      AppIn_BattTemp = [26; 26; 26; 26; 26; 26;];
      AppIn_BattCurrent = 0;
      AppIn_BattVoltages = [4.2; 4.2; 4.2; 4.2; 4.2; 4.2; 4.2; 4.2; 4.2; 4.2; 4.2; 4.2; 4.2; 4.2; 4.2; 4.2; 4.2; 4.2; 4.2; 4.2];
      AppIn_LastStoredSOC = 0;
      AppIn_LastStoredCycle = 0;
      AppIn_I2Cerror = false;
      AppIn_LastStoredSOH = 0;
      AppIn_MachineStatus = VDU_MACHINE_STS_E.VDU_SLEEP;
      AppIn_HVMosfetfb = false;
      AppIn_DCDCMosfetfb = false;
      AppIn_PMosfetfb = false;
      AppIn_BMSVltSnsrFail = false;
      AppIn_BattPackTempSnsrFail = false;
      AppIn_VltImbFlt = false;
      AppIn_TempImbWarn = false;
      AppIn_EEPROMSoCWarn15 = false;
    state step_1
      AppIn_HardwiredIgn = true;
    state step_2
      AppIn_MCUHVIL  = true;
    state step_3
      AppIn_PMosfetfb = true;
    state step_4
      AppIn_LoadVolt = 72;
      AppIn_PackVolt = 75;
    state step_5
      AppIn_HVMosfetfb = true;
    state step_6
      AppIn_DCDCMosfetfb = true;
    state step_7
      AppIn_PMosfetfb = false;
    state step_8
    state step_9
      AppIn_G4T2DischargeFlt = true;
    state step_10
      AppIn_HardwiredIgn = false;
    (default) -> G4T2DischargeToSleep.Run
    G4T2DischargeToSleep.Run -> G4T2DischargeToSleep.step_1
    G4T2DischargeToSleep.step_1 -> G4T2DischargeToSleep.step_2 : [ after(0.2,sec) ]
    G4T2DischargeToSleep.step_2 -> G4T2DischargeToSleep.step_3 : [ after(0.2,sec) ]
    G4T2DischargeToSleep.step_3 -> G4T2DischargeToSleep.step_4 : [ after(0.3,sec) ]
    G4T2DischargeToSleep.step_4 -> G4T2DischargeToSleep.step_5 : [ after(0.2,sec) ]
    G4T2DischargeToSleep.step_5 -> G4T2DischargeToSleep.step_6 : [ after(0.3,sec) ]
    G4T2DischargeToSleep.step_6 -> G4T2DischargeToSleep.step_7 : [ after(0.3,sec) ]
    G4T2DischargeToSleep.step_7 -> G4T2DischargeToSleep.step_8 : [ after(0.3,sec) ]
    G4T2DischargeToSleep.step_8 -> G4T2DischargeToSleep.step_9 : [ after(1,sec) ]
    G4T2DischargeToSleep.step_9 -> G4T2DischargeToSleep.step_10 : [ after(10,sec) ]
  state G4Typ2DischgToSleep
    state Run
      %% Initialize data outputs.
      AppIn_HardwiredIgn = false;
      AppIn_OBCwakeup = OBC_E.Sleep;
      AppIn_RTCwakeup = false;
      AppIn_MCUHVIL = false;
      AppIn_OBCHVIL = false;
      AppIn_SoCLEDSW = false;
      AppIn_ChgMode = Charger_Mode_E.OFF;
      AppIn_CVmodeTimer = CV_Mode_Timer_E.Off;
      AppIn_TRerror = false;
      AppIn_TRtimer = false;
      AppIn_G3CommonFlt = false;
      AppIn_G3DischargeFlt = false;
      AppIn_G4T1DischargeFlt = false;
      AppIn_G4T2DischargeFlt = false;
      AppIn_G4CommonFlt = false;
      AppIn_G4ChargeFlt = false;
      AppIn_OBCHeartbeatFail = false;
      AppIn_LoadVolt = 0;
      AppIn_PackVolt = 0;
      AppIn_ActiveDischg = Active_DisChrg_E.Inactive;
      AppIn_BattTemp = [26; 26; 26; 26; 26; 26;];
      AppIn_BattCurrent = 0;
      AppIn_BattVoltages = [4.2; 4.2; 4.2; 4.2; 4.2; 4.2; 4.2; 4.2; 4.2; 4.2; 4.2; 4.2; 4.2; 4.2; 4.2; 4.2; 4.2; 4.2; 4.2; 4.2];
      AppIn_LastStoredSOC = 0;
      AppIn_LastStoredCycle = 0;
      AppIn_I2Cerror = false;
      AppIn_LastStoredSOH = 0;
      AppIn_MachineStatus = VDU_MACHINE_STS_E.VDU_SLEEP;
      AppIn_HVMosfetfb = false;
      AppIn_DCDCMosfetfb = false;
      AppIn_PMosfetfb = false;
      AppIn_BMSVltSnsrFail = false;
      AppIn_BattPackTempSnsrFail = false;
      AppIn_VltImbFlt = false;
      AppIn_TempImbWarn = false;
      AppIn_EEPROMSoCWarn15 = false;
    state step_1
      AppIn_HardwiredIgn = true;
    state step_2
      AppIn_MCUHVIL  = true;
    state step_3
      AppIn_PMosfetfb = true;
    state step_4
      AppIn_LoadVolt = 72;
      AppIn_PackVolt = 75;
    state step_5
      AppIn_HVMosfetfb = true;
    state step_6
      AppIn_DCDCMosfetfb = true;
    state step_7
      AppIn_PMosfetfb = false;
    state step_8
    state step_9
      AppIn_G4T2DischargeFlt = true;
    state step_10
      AppIn_HardwiredIgn = false;
      AppIn_ActiveDischg = Active_DisChrg_E.Completed;
    (default) -> G4Typ2DischgToSleep.Run
    G4Typ2DischgToSleep.Run -> G4Typ2DischgToSleep.step_1
    G4Typ2DischgToSleep.step_1 -> G4Typ2DischgToSleep.step_2 : [ after(0.2,sec) ]
    G4Typ2DischgToSleep.step_2 -> G4Typ2DischgToSleep.step_3 : [ after(0.2,sec) ]
    G4Typ2DischgToSleep.step_3 -> G4Typ2DischgToSleep.step_4 : [ after(0.3,sec) ]
    G4Typ2DischgToSleep.step_4 -> G4Typ2DischgToSleep.step_5 : [ after(0.2,sec) ]
    G4Typ2DischgToSleep.step_5 -> G4Typ2DischgToSleep.step_6 : [ after(0.3,sec) ]
    G4Typ2DischgToSleep.step_6 -> G4Typ2DischgToSleep.step_7 : [ after(0.3,sec) ]
    G4Typ2DischgToSleep.step_7 -> G4Typ2DischgToSleep.step_8 : [ after(0.3,sec) ]
    G4Typ2DischgToSleep.step_8 -> G4Typ2DischgToSleep.step_9 : [ after(1,sec) ]
    G4Typ2DischgToSleep.step_9 -> G4Typ2DischgToSleep.step_10 : [ after(6,sec) ]
  state G4T1DischargeToSleep
    state Run
      %% Initialize data outputs.
      AppIn_HardwiredIgn = false;
      AppIn_OBCwakeup = OBC_E.Sleep;
      AppIn_RTCwakeup = false;
      AppIn_MCUHVIL = false;
      AppIn_OBCHVIL = false;
      AppIn_SoCLEDSW = false;
      AppIn_ChgMode = Charger_Mode_E.OFF;
      AppIn_CVmodeTimer = CV_Mode_Timer_E.Off;
      AppIn_TRerror = false;
      AppIn_TRtimer = false;
      AppIn_G3CommonFlt = false;
      AppIn_G3DischargeFlt = false;
      AppIn_G4T1DischargeFlt = false;
      AppIn_G4T2DischargeFlt = false;
      AppIn_G4CommonFlt = false;
      AppIn_G4ChargeFlt = false;
      AppIn_OBCHeartbeatFail = false;
      AppIn_LoadVolt = 0;
      AppIn_PackVolt = 0;
      AppIn_ActiveDischg = Active_DisChrg_E.Inactive;
      AppIn_BattTemp = [26; 26; 26; 26; 26; 26;];
      AppIn_BattCurrent = 0;
      AppIn_BattVoltages = [4.2; 4.2; 4.2; 4.2; 4.2; 4.2; 4.2; 4.2; 4.2; 4.2; 4.2; 4.2; 4.2; 4.2; 4.2; 4.2; 4.2; 4.2; 4.2; 4.2];
      AppIn_LastStoredSOC = 0;
      AppIn_LastStoredCycle = 0;
      AppIn_I2Cerror = false;
      AppIn_LastStoredSOH = 0;
      AppIn_MachineStatus = VDU_MACHINE_STS_E.VDU_SLEEP;
      AppIn_HVMosfetfb = false;
      AppIn_DCDCMosfetfb = false;
      AppIn_PMosfetfb = false;
      AppIn_BMSVltSnsrFail = false;
      AppIn_BattPackTempSnsrFail = false;
      AppIn_VltImbFlt = false;
      AppIn_TempImbWarn = false;
      AppIn_EEPROMSoCWarn15 = false;
    state step_1
      AppIn_HardwiredIgn = true;
    state step_2
      AppIn_MCUHVIL  = true;
    state step_3
      AppIn_PMosfetfb = true;
    state step_4
      AppIn_LoadVolt = 72;
      AppIn_PackVolt = 75;
    state step_5
      AppIn_HVMosfetfb = true;
    state step_6
      AppIn_DCDCMosfetfb = true;
    state step_7
      AppIn_PMosfetfb = false;
    state step_8
    state step_9
      AppIn_G4T1DischargeFlt = true;
    state step_10
      AppIn_HardwiredIgn = false;
    (default) -> G4T1DischargeToSleep.Run
    G4T1DischargeToSleep.Run -> G4T1DischargeToSleep.step_1
    G4T1DischargeToSleep.step_1 -> G4T1DischargeToSleep.step_2 : [ after(0.2,sec) ]
    G4T1DischargeToSleep.step_2 -> G4T1DischargeToSleep.step_3 : [ after(0.2,sec) ]
    G4T1DischargeToSleep.step_3 -> G4T1DischargeToSleep.step_4 : [ after(0.3,sec) ]
    G4T1DischargeToSleep.step_4 -> G4T1DischargeToSleep.step_5 : [ after(0.2,sec) ]
    G4T1DischargeToSleep.step_5 -> G4T1DischargeToSleep.step_6 : [ after(0.3,sec) ]
    G4T1DischargeToSleep.step_6 -> G4T1DischargeToSleep.step_7 : [ after(0.3,sec) ]
    G4T1DischargeToSleep.step_7 -> G4T1DischargeToSleep.step_8 : [ after(0.3,sec) ]
    G4T1DischargeToSleep.step_8 -> G4T1DischargeToSleep.step_9 : [ after(1,sec) ]
    G4T1DischargeToSleep.step_9 -> G4T1DischargeToSleep.step_10 : [ after(10,sec) ]
  state G4Typ1DischgToSleep
    state Run
      %% Initialize data outputs.
      AppIn_HardwiredIgn = false;
      AppIn_OBCwakeup = OBC_E.Sleep;
      AppIn_RTCwakeup = false;
      AppIn_MCUHVIL = false;
      AppIn_OBCHVIL = false;
      AppIn_SoCLEDSW = false;
      AppIn_ChgMode = Charger_Mode_E.OFF;
      AppIn_CVmodeTimer = CV_Mode_Timer_E.Off;
      AppIn_TRerror = false;
      AppIn_TRtimer = false;
      AppIn_G3CommonFlt = false;
      AppIn_G3DischargeFlt = false;
      AppIn_G4T1DischargeFlt = false;
      AppIn_G4T2DischargeFlt = false;
      AppIn_G4CommonFlt = false;
      AppIn_G4ChargeFlt = false;
      AppIn_OBCHeartbeatFail = false;
      AppIn_LoadVolt = 0;
      AppIn_PackVolt = 0;
      AppIn_ActiveDischg = Active_DisChrg_E.Inactive;
      AppIn_BattTemp = [26; 26; 26; 26; 26; 26;];
      AppIn_BattCurrent = 0;
      AppIn_BattVoltages = [4.2; 4.2; 4.2; 4.2; 4.2; 4.2; 4.2; 4.2; 4.2; 4.2; 4.2; 4.2; 4.2; 4.2; 4.2; 4.2; 4.2; 4.2; 4.2; 4.2];
      AppIn_LastStoredSOC = 0;
      AppIn_LastStoredCycle = 0;
      AppIn_I2Cerror = false;
      AppIn_LastStoredSOH = 0;
      AppIn_MachineStatus = VDU_MACHINE_STS_E.VDU_SLEEP;
      AppIn_HVMosfetfb = false;
      AppIn_DCDCMosfetfb = false;
      AppIn_PMosfetfb = false;
      AppIn_BMSVltSnsrFail = false;
      AppIn_BattPackTempSnsrFail = false;
      AppIn_VltImbFlt = false;
      AppIn_TempImbWarn = false;
      AppIn_EEPROMSoCWarn15 = false;
    state step_1
      AppIn_HardwiredIgn = true;
    state step_2
      AppIn_MCUHVIL  = true;
    state step_3
      AppIn_PMosfetfb = true;
    state step_4
      AppIn_LoadVolt = 72;
      AppIn_PackVolt = 75;
    state step_5
      AppIn_HVMosfetfb = true;
    state step_6
      AppIn_DCDCMosfetfb = true;
    state step_7
      AppIn_PMosfetfb = false;
    state step_8
    state step_9
      AppIn_G4T1DischargeFlt = true;
    state step_10
      AppIn_HardwiredIgn = false;
      AppIn_ActiveDischg = Active_DisChrg_E.Completed;
    (default) -> G4Typ1DischgToSleep.Run
    G4Typ1DischgToSleep.Run -> G4Typ1DischgToSleep.step_1
    G4Typ1DischgToSleep.step_1 -> G4Typ1DischgToSleep.step_2 : [ after(0.2,sec) ]
    G4Typ1DischgToSleep.step_2 -> G4Typ1DischgToSleep.step_3 : [ after(0.2,sec) ]
    G4Typ1DischgToSleep.step_3 -> G4Typ1DischgToSleep.step_4 : [ after(0.3,sec) ]
    G4Typ1DischgToSleep.step_4 -> G4Typ1DischgToSleep.step_5 : [ after(0.2,sec) ]
    G4Typ1DischgToSleep.step_5 -> G4Typ1DischgToSleep.step_6 : [ after(0.3,sec) ]
    G4Typ1DischgToSleep.step_6 -> G4Typ1DischgToSleep.step_7 : [ after(0.3,sec) ]
    G4Typ1DischgToSleep.step_7 -> G4Typ1DischgToSleep.step_8 : [ after(0.3,sec) ]
    G4Typ1DischgToSleep.step_8 -> G4Typ1DischgToSleep.step_9 : [ after(1,sec) ]
    G4Typ1DischgToSleep.step_9 -> G4Typ1DischgToSleep.step_10 : [ after(6,sec) ]
  state G4CommonToSleep
    state Run
      %% Initialize data outputs.
      AppIn_HardwiredIgn = false;
      AppIn_OBCwakeup = OBC_E.Sleep;
      AppIn_RTCwakeup = false;
      AppIn_MCUHVIL = false;
      AppIn_OBCHVIL = false;
      AppIn_SoCLEDSW = false;
      AppIn_ChgMode = Charger_Mode_E.OFF;
      AppIn_CVmodeTimer = CV_Mode_Timer_E.Off;
      AppIn_TRerror = false;
      AppIn_TRtimer = false;
      AppIn_G3CommonFlt = false;
      AppIn_G3DischargeFlt = false;
      AppIn_G4T1DischargeFlt = false;
      AppIn_G4T2DischargeFlt = false;
      AppIn_G4CommonFlt = false;
      AppIn_G4ChargeFlt = false;
      AppIn_OBCHeartbeatFail = false;
      AppIn_LoadVolt = 0;
      AppIn_PackVolt = 0;
      AppIn_ActiveDischg = Active_DisChrg_E.Inactive;
      AppIn_BattTemp = [26; 26; 26; 26; 26; 26;];
      AppIn_BattCurrent = 0;
      AppIn_BattVoltages = [4.2; 4.2; 4.2; 4.2; 4.2; 4.2; 4.2; 4.2; 4.2; 4.2; 4.2; 4.2; 4.2; 4.2; 4.2; 4.2; 4.2; 4.2; 4.2; 4.2];
      AppIn_LastStoredSOC = 0;
      AppIn_LastStoredCycle = 0;
      AppIn_I2Cerror = false;
      AppIn_LastStoredSOH = 0;
      AppIn_MachineStatus = VDU_MACHINE_STS_E.VDU_SLEEP;
      AppIn_HVMosfetfb = false;
      AppIn_DCDCMosfetfb = false;
      AppIn_PMosfetfb = false;
      AppIn_BMSVltSnsrFail = false;
      AppIn_BattPackTempSnsrFail = false;
      AppIn_VltImbFlt = false;
      AppIn_TempImbWarn = false;
      AppIn_EEPROMSoCWarn15 = false;
    state step_1
      AppIn_HardwiredIgn = true;
    state step_2
      AppIn_MCUHVIL  = true;
    state step_3
      AppIn_PMosfetfb = true;
    state step_4
      AppIn_LoadVolt = 72;
      AppIn_PackVolt = 75;
    state step_5
      AppIn_HVMosfetfb = true;
    state step_6
      AppIn_DCDCMosfetfb = true;
    state step_7
      AppIn_PMosfetfb = false;
    state step_8
    state step_9
      AppIn_G4CommonFlt = true;
    state step_10
      AppIn_HardwiredIgn = false;
    (default) -> G4CommonToSleep.Run
    G4CommonToSleep.Run -> G4CommonToSleep.step_1
    G4CommonToSleep.step_1 -> G4CommonToSleep.step_2 : [ after(0.2,sec) ]
    G4CommonToSleep.step_2 -> G4CommonToSleep.step_3 : [ after(0.2,sec) ]
    G4CommonToSleep.step_3 -> G4CommonToSleep.step_4 : [ after(0.3,sec) ]
    G4CommonToSleep.step_4 -> G4CommonToSleep.step_5 : [ after(0.2,sec) ]
    G4CommonToSleep.step_5 -> G4CommonToSleep.step_6 : [ after(0.3,sec) ]
    G4CommonToSleep.step_6 -> G4CommonToSleep.step_7 : [ after(0.3,sec) ]
    G4CommonToSleep.step_7 -> G4CommonToSleep.step_8 : [ after(0.3,sec) ]
    G4CommonToSleep.step_8 -> G4CommonToSleep.step_9 : [ after(1,sec) ]
    G4CommonToSleep.step_9 -> G4CommonToSleep.step_10 : [ after(10,sec) ]
  state G4CommToSleep
    state Run
      %% Initialize data outputs.
      AppIn_HardwiredIgn = false;
      AppIn_OBCwakeup = OBC_E.Sleep;
      AppIn_RTCwakeup = false;
      AppIn_MCUHVIL = false;
      AppIn_OBCHVIL = false;
      AppIn_SoCLEDSW = false;
      AppIn_ChgMode = Charger_Mode_E.OFF;
      AppIn_CVmodeTimer = CV_Mode_Timer_E.Off;
      AppIn_TRerror = false;
      AppIn_TRtimer = false;
      AppIn_G3CommonFlt = false;
      AppIn_G3DischargeFlt = false;
      AppIn_G4T1DischargeFlt = false;
      AppIn_G4T2DischargeFlt = false;
      AppIn_G4CommonFlt = false;
      AppIn_G4ChargeFlt = false;
      AppIn_OBCHeartbeatFail = false;
      AppIn_LoadVolt = 0;
      AppIn_PackVolt = 0;
      AppIn_ActiveDischg = Active_DisChrg_E.Inactive;
      AppIn_BattTemp = [26; 26; 26; 26; 26; 26;];
      AppIn_BattCurrent = 0;
      AppIn_BattVoltages = [4.2; 4.2; 4.2; 4.2; 4.2; 4.2; 4.2; 4.2; 4.2; 4.2; 4.2; 4.2; 4.2; 4.2; 4.2; 4.2; 4.2; 4.2; 4.2; 4.2];
      AppIn_LastStoredSOC = 0;
      AppIn_LastStoredCycle = 0;
      AppIn_I2Cerror = false;
      AppIn_LastStoredSOH = 0;
      AppIn_MachineStatus = VDU_MACHINE_STS_E.VDU_SLEEP;
      AppIn_HVMosfetfb = false;
      AppIn_DCDCMosfetfb = false;
      AppIn_PMosfetfb = false;
      AppIn_BMSVltSnsrFail = false;
      AppIn_BattPackTempSnsrFail = false;
      AppIn_VltImbFlt = false;
      AppIn_TempImbWarn = false;
      AppIn_EEPROMSoCWarn15 = false;
    state step_1
      AppIn_HardwiredIgn = true;
    state step_2
      AppIn_MCUHVIL  = true;
    state step_3
      AppIn_PMosfetfb = true;
    state step_4
      AppIn_LoadVolt = 72;
      AppIn_PackVolt = 75;
    state step_5
      AppIn_HVMosfetfb = true;
    state step_6
      AppIn_DCDCMosfetfb = true;
    state step_7
      AppIn_PMosfetfb = false;
    state step_8
    state step_9
      AppIn_G4CommonFlt = true;
    state step_10
      AppIn_HardwiredIgn = false;
    state step_11
      AppIn_ActiveDischg = Active_DisChrg_E.Completed;
    (default) -> G4CommToSleep.Run
    G4CommToSleep.Run -> G4CommToSleep.step_1
    G4CommToSleep.step_1 -> G4CommToSleep.step_2 : [ after(0.2,sec) ]
    G4CommToSleep.step_2 -> G4CommToSleep.step_3 : [ after(0.2,sec) ]
    G4CommToSleep.step_3 -> G4CommToSleep.step_4 : [ after(0.3,sec) ]
    G4CommToSleep.step_4 -> G4CommToSleep.step_5 : [ after(0.2,sec) ]
    G4CommToSleep.step_5 -> G4CommToSleep.step_6 : [ after(0.3,sec) ]
    G4CommToSleep.step_6 -> G4CommToSleep.step_7 : [ after(0.3,sec) ]
    G4CommToSleep.step_7 -> G4CommToSleep.step_8 : [ after(0.3,sec) ]
    G4CommToSleep.step_8 -> G4CommToSleep.step_9 : [ after(1,sec) ]
    G4CommToSleep.step_9 -> G4CommToSleep.step_10 : [ after(6,sec) ]
    G4CommToSleep.step_10 -> G4CommToSleep.step_11 : [ after(0.1,sec) ]
  state G4ChargeToSleep
    state Run
      %% Initialize data outputs.
      AppIn_HardwiredIgn = false;
      AppIn_OBCwakeup = OBC_E.Sleep;
      AppIn_RTCwakeup = false;
      AppIn_MCUHVIL = false;
      AppIn_OBCHVIL = false;
      AppIn_SoCLEDSW = false;
      AppIn_ChgMode = Charger_Mode_E.OFF;
      AppIn_CVmodeTimer = CV_Mode_Timer_E.Off;
      AppIn_TRerror = false;
      AppIn_TRtimer = false;
      AppIn_G3CommonFlt = false;
      AppIn_G3DischargeFlt = false;
      AppIn_G4T1DischargeFlt = false;
      AppIn_G4T2DischargeFlt = false;
      AppIn_G4CommonFlt = false;
      AppIn_G4ChargeFlt = false;
      AppIn_OBCHeartbeatFail = false;
      AppIn_LoadVolt = 0;
      AppIn_PackVolt = 0;
      AppIn_ActiveDischg = Active_DisChrg_E.Inactive;
      AppIn_BattTemp = [26; 26; 26; 26; 26; 26;];
      AppIn_BattCurrent = 0;
      AppIn_BattVoltages = [4.2; 4.2; 4.2; 4.2; 4.2; 4.2; 4.2; 4.2; 4.2; 4.2; 4.2; 4.2; 4.2; 4.2; 4.2; 4.2; 4.2; 4.2; 4.2; 4.2];
      AppIn_LastStoredSOC = 0;
      AppIn_LastStoredCycle = 0;
      AppIn_I2Cerror = false;
      AppIn_LastStoredSOH = 0;
      AppIn_MachineStatus = VDU_MACHINE_STS_E.VDU_SLEEP;
      AppIn_HVMosfetfb = false;
      AppIn_DCDCMosfetfb = false;
      AppIn_PMosfetfb = false;
      AppIn_BMSVltSnsrFail = false;
      AppIn_BattPackTempSnsrFail = false;
      AppIn_VltImbFlt = false;
      AppIn_TempImbWarn = false;
      AppIn_EEPROMSoCWarn15 = false;
    state step_1
      AppIn_HardwiredIgn = true;
    state step_2
      AppIn_OBCwakeup = OBC_E.Wake_Up;
      AppIn_OBCHVIL= true;
    state step_3
      AppIn_PMosfetfb = true;
    state step_4
      AppIn_LoadVolt = 72;
      AppIn_PackVolt = 75;
    state step_5
      AppIn_HVMosfetfb = true;
    state step_6
      AppIn_DCDCMosfetfb = true;
    state step_7
      AppIn_PMosfetfb = false;
    state step_8
    state step_9
      AppIn_G4ChargeFlt = true;
    state step_10
      AppIn_HardwiredIgn = false;
      AppIn_OBCwakeup = OBC_E.Sleep;
    (default) -> G4ChargeToSleep.Run
    G4ChargeToSleep.Run -> G4ChargeToSleep.step_1
    G4ChargeToSleep.step_1 -> G4ChargeToSleep.step_2 : [ after(0.2,sec) ]
    G4ChargeToSleep.step_2 -> G4ChargeToSleep.step_3 : [ after(0.2,sec) ]
    G4ChargeToSleep.step_3 -> G4ChargeToSleep.step_4 : [ after(0.3,sec) ]
    G4ChargeToSleep.step_4 -> G4ChargeToSleep.step_5 : [ after(0.2,sec) ]
    G4ChargeToSleep.step_5 -> G4ChargeToSleep.step_6 : [ after(0.3,sec) ]
    G4ChargeToSleep.step_6 -> G4ChargeToSleep.step_7 : [ after(0.3,sec) ]
    G4ChargeToSleep.step_7 -> G4ChargeToSleep.step_8 : [ after(0.3,sec) ]
    G4ChargeToSleep.step_8 -> G4ChargeToSleep.step_9 : [ after(1,sec) ]
    G4ChargeToSleep.step_9 -> G4ChargeToSleep.step_10 : [ after(10,sec) ]
  state G4ChgToSleep
    state Run
      %% Initialize data outputs.
      AppIn_HardwiredIgn = false;
      AppIn_OBCwakeup = OBC_E.Sleep;
      AppIn_RTCwakeup = false;
      AppIn_MCUHVIL = false;
      AppIn_OBCHVIL = false;
      AppIn_SoCLEDSW = false;
      AppIn_ChgMode = Charger_Mode_E.OFF;
      AppIn_CVmodeTimer = CV_Mode_Timer_E.Off;
      AppIn_TRerror = false;
      AppIn_TRtimer = false;
      AppIn_G3CommonFlt = false;
      AppIn_G3DischargeFlt = false;
      AppIn_G4T1DischargeFlt = false;
      AppIn_G4T2DischargeFlt = false;
      AppIn_G4CommonFlt = false;
      AppIn_G4ChargeFlt = false;
      AppIn_OBCHeartbeatFail = false;
      AppIn_LoadVolt = 0;
      AppIn_PackVolt = 0;
      AppIn_ActiveDischg = Active_DisChrg_E.Inactive;
      AppIn_BattTemp = [26; 26; 26; 26; 26; 26;];
      AppIn_BattCurrent = 0;
      AppIn_BattVoltages = [4.2; 4.2; 4.2; 4.2; 4.2; 4.2; 4.2; 4.2; 4.2; 4.2; 4.2; 4.2; 4.2; 4.2; 4.2; 4.2; 4.2; 4.2; 4.2; 4.2];
      AppIn_LastStoredSOC = 0;
      AppIn_LastStoredCycle = 0;
      AppIn_I2Cerror = false;
      AppIn_LastStoredSOH = 0;
      AppIn_MachineStatus = VDU_MACHINE_STS_E.VDU_SLEEP;
      AppIn_HVMosfetfb = false;
      AppIn_DCDCMosfetfb = false;
      AppIn_PMosfetfb = false;
      AppIn_BMSVltSnsrFail = false;
      AppIn_BattPackTempSnsrFail = false;
      AppIn_VltImbFlt = false;
      AppIn_TempImbWarn = false;
      AppIn_EEPROMSoCWarn15 = false;
    state step_1
      AppIn_HardwiredIgn = true;
    state step_2
      AppIn_OBCwakeup = OBC_E.Wake_Up;
      AppIn_OBCHVIL= true;
    state step_3
      AppIn_PMosfetfb = true;
    state step_4
      AppIn_LoadVolt = 72;
      AppIn_PackVolt = 75;
    state step_5
      AppIn_HVMosfetfb = true;
    state step_6
      AppIn_DCDCMosfetfb = true;
    state step_7
      AppIn_PMosfetfb = false;
    state step_8
    state step_9
      AppIn_G4ChargeFlt = true;
    state step_10
      AppIn_OBCwakeup = OBC_E.Sleep;
      AppIn_HardwiredIgn = false;
      AppIn_ActiveDischg = Active_DisChrg_E.Completed;
    (default) -> G4ChgToSleep.Run
    G4ChgToSleep.Run -> G4ChgToSleep.step_1
    G4ChgToSleep.step_1 -> G4ChgToSleep.step_2 : [ after(0.2,sec) ]
    G4ChgToSleep.step_2 -> G4ChgToSleep.step_3 : [ after(0.2,sec) ]
    G4ChgToSleep.step_3 -> G4ChgToSleep.step_4 : [ after(0.3,sec) ]
    G4ChgToSleep.step_4 -> G4ChgToSleep.step_5 : [ after(0.2,sec) ]
    G4ChgToSleep.step_5 -> G4ChgToSleep.step_6 : [ after(0.3,sec) ]
    G4ChgToSleep.step_6 -> G4ChgToSleep.step_7 : [ after(0.3,sec) ]
    G4ChgToSleep.step_7 -> G4ChgToSleep.step_8 : [ after(0.3,sec) ]
    G4ChgToSleep.step_8 -> G4ChgToSleep.step_9 : [ after(1,sec) ]
    G4ChgToSleep.step_9 -> G4ChgToSleep.step_10 : [ after(6,sec) ]
  state ChgToDischgToChg
    state Run
      %% Initialize data outputs.
      AppIn_HardwiredIgn = false;
      AppIn_OBCwakeup = OBC_E.Sleep;
      AppIn_RTCwakeup = false;
      AppIn_MCUHVIL = false;
      AppIn_OBCHVIL = false;
      AppIn_SoCLEDSW = false;
      AppIn_ChgMode = Charger_Mode_E.OFF;
      AppIn_CVmodeTimer = CV_Mode_Timer_E.Off;
      AppIn_TRerror = false;
      AppIn_TRtimer = false;
      AppIn_G3CommonFlt = false;
      AppIn_G3DischargeFlt = false;
      AppIn_G4T1DischargeFlt = false;
      AppIn_G4T2DischargeFlt = false;
      AppIn_G4CommonFlt = false;
      AppIn_G4ChargeFlt = false;
      AppIn_OBCHeartbeatFail = false;
      AppIn_LoadVolt = 0;
      AppIn_PackVolt = 0;
      AppIn_ActiveDischg = Active_DisChrg_E.Inactive;
      AppIn_BattTemp = [26; 26; 26; 26; 26; 26;];
      AppIn_BattCurrent = 0;
      AppIn_BattVoltages = [4.2; 4.2; 4.2; 4.2; 4.2; 4.2; 4.2; 4.2; 4.2; 4.2; 4.2; 4.2; 4.2; 4.2; 4.2; 4.2; 4.2; 4.2; 4.2; 4.2];
      AppIn_LastStoredSOC = 0;
      AppIn_LastStoredCycle = 0;
      AppIn_I2Cerror = false;
      AppIn_LastStoredSOH = 0;
      AppIn_MachineStatus = VDU_MACHINE_STS_E.VDU_SLEEP;
      AppIn_HVMosfetfb = false;
      AppIn_DCDCMosfetfb = false;
      AppIn_PMosfetfb = false;
      AppIn_BMSVltSnsrFail = false;
      AppIn_BattPackTempSnsrFail = false;
      AppIn_VltImbFlt = false;
      AppIn_TempImbWarn = false;
      AppIn_EEPROMSoCWarn15 = false;
    state step_1
      AppIn_HardwiredIgn = true;
    state step_2
      AppIn_OBCwakeup = OBC_E.Wake_Up;
      AppIn_OBCHVIL= true;
    state step_3
      AppIn_PMosfetfb = true;
    state step_4
      AppIn_LoadVolt = 72;
      AppIn_PackVolt = 75;
    state step_5
      AppIn_HVMosfetfb = true;
    state step_6
      AppIn_DCDCMosfetfb = true;
    state step_7
      AppIn_PMosfetfb = false;
    state step_8
    state step_9
      AppIn_OBCHVIL= false;
      AppIn_OBCwakeup = OBC_E.Sleep;
    state step_10
      AppIn_MCUHVIL  = true;
    state step_11
      AppIn_HardwiredIgn = false;
      AppIn_HVMosfetfb = false;
    (default) -> ChgToDischgToChg.Run
    ChgToDischgToChg.Run -> ChgToDischgToChg.step_1
    ChgToDischgToChg.step_1 -> ChgToDischgToChg.step_2 : [ after(0.2,sec) ]
    ChgToDischgToChg.step_2 -> ChgToDischgToChg.step_3 : [ after(0.5,sec) ]
    ChgToDischgToChg.step_3 -> ChgToDischgToChg.step_4 : [ after(0.5,sec) ]
    ChgToDischgToChg.step_4 -> ChgToDischgToChg.step_5 : [ after(0.2,sec) ]
    ChgToDischgToChg.step_5 -> ChgToDischgToChg.step_6 : [ after(0.5,sec) ]
    ChgToDischgToChg.step_6 -> ChgToDischgToChg.step_7 : [ after(0.5,sec) ]
    ChgToDischgToChg.step_7 -> ChgToDischgToChg.step_8 : [ after(0.5,sec) ]
    ChgToDischgToChg.step_8 -> ChgToDischgToChg.step_9 : [ after(1,sec) ]
    ChgToDischgToChg.step_9 -> ChgToDischgToChg.step_10 : [ after(0.2,sec) ]
    ChgToDischgToChg.step_10 -> ChgToDischgToChg.step_11 : [ after(0.5,sec) ]
  state G4CommFltToChg
    state Run
      %% Initialize data outputs.
      AppIn_HardwiredIgn = false;
      AppIn_OBCwakeup = OBC_E.Sleep;
      AppIn_RTCwakeup = false;
      AppIn_MCUHVIL = false;
      AppIn_OBCHVIL = false;
      AppIn_SoCLEDSW = false;
      AppIn_ChgMode = Charger_Mode_E.OFF;
      AppIn_CVmodeTimer = CV_Mode_Timer_E.Off;
      AppIn_TRerror = false;
      AppIn_TRtimer = false;
      AppIn_G3CommonFlt = false;
      AppIn_G3DischargeFlt = false;
      AppIn_G4T1DischargeFlt = false;
      AppIn_G4T2DischargeFlt = false;
      AppIn_G4CommonFlt = false;
      AppIn_G4ChargeFlt = false;
      AppIn_OBCHeartbeatFail = false;
      AppIn_LoadVolt = 0;
      AppIn_PackVolt = 0;
      AppIn_ActiveDischg = Active_DisChrg_E.Inactive;
      AppIn_BattTemp = [26; 26; 26; 26; 26; 26;];
      AppIn_BattCurrent = 0;
      AppIn_BattVoltages = [4.2; 4.2; 4.2; 4.2; 4.2; 4.2; 4.2; 4.2; 4.2; 4.2; 4.2; 4.2; 4.2; 4.2; 4.2; 4.2; 4.2; 4.2; 4.2; 4.2];
      AppIn_LastStoredSOC = 0;
      AppIn_LastStoredCycle = 0;
      AppIn_I2Cerror = false;
      AppIn_LastStoredSOH = 0;
      AppIn_MachineStatus = VDU_MACHINE_STS_E.VDU_SLEEP;
      AppIn_HVMosfetfb = false;
      AppIn_DCDCMosfetfb = false;
      AppIn_PMosfetfb = false;
      AppIn_BMSVltSnsrFail = false;
      AppIn_BattPackTempSnsrFail = false;
      AppIn_VltImbFlt = false;
      AppIn_TempImbWarn = false;
      AppIn_EEPROMSoCWarn15 = false;
    state step_1
      AppIn_HardwiredIgn = true;
    state step_2
      AppIn_MCUHVIL  = true;
    state step_3
      AppIn_PMosfetfb = true;
    state step_4
      AppIn_LoadVolt = 72;
      AppIn_PackVolt = 75;
    state step_5
      AppIn_HVMosfetfb = true;
    state step_6
      AppIn_DCDCMosfetfb = true;
    state step_7
      AppIn_PMosfetfb = false;
    state step_8
    state step_9
      AppIn_G4CommonFlt = true;
    state step_10
      AppIn_HardwiredIgn = false;
    state step_11
      AppIn_G4CommonFlt = false;
      AppIn_OBCwakeup = OBC_E.Wake_Up;
      AppIn_OBCHVIL= true;
    state step_12
      AppIn_PMosfetfb = true;
    state step_13
      AppIn_HVMosfetfb = true;
    state step_14
      AppIn_DCDCMosfetfb = false;
    state step_15
      AppIn_PMosfetfb = false;
    state step_16
    (default) -> G4CommFltToChg.Run
    G4CommFltToChg.Run -> G4CommFltToChg.step_1
    G4CommFltToChg.step_1 -> G4CommFltToChg.step_2 : [ after(0.2,sec) ]
    G4CommFltToChg.step_2 -> G4CommFltToChg.step_3 : [ after(0.2,sec) ]
    G4CommFltToChg.step_3 -> G4CommFltToChg.step_4 : [ after(0.3,sec) ]
    G4CommFltToChg.step_4 -> G4CommFltToChg.step_5 : [ after(0.2,sec) ]
    G4CommFltToChg.step_5 -> G4CommFltToChg.step_6 : [ after(0.3,sec) ]
    G4CommFltToChg.step_6 -> G4CommFltToChg.step_7 : [ after(0.3,sec) ]
    G4CommFltToChg.step_7 -> G4CommFltToChg.step_8 : [ after(0.3,sec) ]
    G4CommFltToChg.step_8 -> G4CommFltToChg.step_9 : [ after(1,sec) ]
    G4CommFltToChg.step_9 -> G4CommFltToChg.step_10 : [ after(6,sec) ]
    G4CommFltToChg.step_10 -> G4CommFltToChg.step_11 : [ after(0.2,sec) ]
    G4CommFltToChg.step_11 -> G4CommFltToChg.step_12 : [ after(0.2,sec) ]
    G4CommFltToChg.step_12 -> G4CommFltToChg.step_13 : [ after(0.4,sec) ]
    G4CommFltToChg.step_13 -> G4CommFltToChg.step_14 : [ after(0.3,sec) ]
    G4CommFltToChg.step_14 -> G4CommFltToChg.step_15 : [ after(0.3,sec) ]
    G4CommFltToChg.step_15 -> G4CommFltToChg.step_16 : [ after(1,sec) ]
  state G4ChgFltToDischg
    state Run
      %% Initialize data outputs.
      AppIn_HardwiredIgn = false;
      AppIn_OBCwakeup = OBC_E.Sleep;
      AppIn_RTCwakeup = false;
      AppIn_MCUHVIL = true;
      AppIn_OBCHVIL = false;
      AppIn_SoCLEDSW = false;
      AppIn_ChgMode = Charger_Mode_E.OFF;
      AppIn_CVmodeTimer = CV_Mode_Timer_E.Off;
      AppIn_TRerror = false;
      AppIn_TRtimer = false;
      AppIn_G3CommonFlt = false;
      AppIn_G3DischargeFlt = false;
      AppIn_G4T1DischargeFlt = false;
      AppIn_G4T2DischargeFlt = false;
      AppIn_G4CommonFlt = false;
      AppIn_G4ChargeFlt = false;
      AppIn_OBCHeartbeatFail = false;
      AppIn_LoadVolt = 0;
      AppIn_PackVolt = 0;
      AppIn_ActiveDischg = Active_DisChrg_E.Inactive;
      AppIn_BattTemp = [26; 26; 26; 26; 26; 26;];
      AppIn_BattCurrent = 0;
      AppIn_BattVoltages = [4.2; 4.2; 4.2; 4.2; 4.2; 4.2; 4.2; 4.2; 4.2; 4.2; 4.2; 4.2; 4.2; 4.2; 4.2; 4.2; 4.2; 4.2; 4.2; 4.2];
      AppIn_LastStoredSOC = 0;
      AppIn_LastStoredCycle = 0;
      AppIn_I2Cerror = false;
      AppIn_LastStoredSOH = 0;
      AppIn_MachineStatus = VDU_MACHINE_STS_E.VDU_SLEEP;
      AppIn_HVMosfetfb = false;
      AppIn_DCDCMosfetfb = false;
      AppIn_PMosfetfb = false;
      AppIn_BMSVltSnsrFail = false;
      AppIn_BattPackTempSnsrFail = false;
      AppIn_VltImbFlt = false;
      AppIn_TempImbWarn = false;
      AppIn_EEPROMSoCWarn15 = false;
    state step_1
      AppIn_OBCwakeup = OBC_E.Wake_Up;
      AppIn_OBCHVIL= true;
    state step_2
      AppIn_PMosfetfb = true;
    state step_3
      AppIn_LoadVolt = 72;
      AppIn_PackVolt = 75;
    state step_4
      AppIn_HVMosfetfb = true;
    state step_5
      AppIn_PMosfetfb = false;
    state step_6
    state step_7
      AppIn_G4ChargeFlt = true;
    state step_8
      AppIn_G4ChargeFlt = false;
      AppIn_HardwiredIgn = true;
      AppIn_OBCwakeup = OBC_E.Sleep;
      AppIn_OBCHVIL= false;
    state step_9
      AppIn_PMosfetfb = true;
    state step_10
      AppIn_HVMosfetfb = true;
    state step_11
      AppIn_DCDCMosfetfb = true;
    state step_12
      AppIn_PMosfetfb = false;
    (default) -> G4ChgFltToDischg.Run
    G4ChgFltToDischg.Run -> G4ChgFltToDischg.step_1
    G4ChgFltToDischg.step_1 -> G4ChgFltToDischg.step_2 : [ after(0.2,sec) ]
    G4ChgFltToDischg.step_2 -> G4ChgFltToDischg.step_3 : [ after(0.3,sec) ]
    G4ChgFltToDischg.step_3 -> G4ChgFltToDischg.step_4 : [ after(0.2,sec) ]
    G4ChgFltToDischg.step_4 -> G4ChgFltToDischg.step_5 : [ after(0.5,sec) ]
    G4ChgFltToDischg.step_5 -> G4ChgFltToDischg.step_6 : [ after(0.3,sec) ]
    G4ChgFltToDischg.step_6 -> G4ChgFltToDischg.step_7 : [ after(1,sec) ]
    G4ChgFltToDischg.step_7 -> G4ChgFltToDischg.step_8 : [ after(6,sec) ]
    G4ChgFltToDischg.step_8 -> G4ChgFltToDischg.step_9 : [ after(0.2,sec) ]
    G4ChgFltToDischg.step_9 -> G4ChgFltToDischg.step_10 : [ after(0.3,sec) ]
    G4ChgFltToDischg.step_10 -> G4ChgFltToDischg.step_11 : [ after(0.3,sec) ]
    G4ChgFltToDischg.step_11 -> G4ChgFltToDischg.step_12 : [ after(0.3,sec) ]
  state G4T1DischgToG4T2Dischg
    state Run
      %% Initialize data outputs.
      AppIn_HardwiredIgn = false;
      AppIn_OBCwakeup = OBC_E.Sleep;
      AppIn_RTCwakeup = false;
      AppIn_MCUHVIL = false;
      AppIn_OBCHVIL = false;
      AppIn_SoCLEDSW = false;
      AppIn_ChgMode = Charger_Mode_E.OFF;
      AppIn_CVmodeTimer = CV_Mode_Timer_E.Off;
      AppIn_TRerror = false;
      AppIn_TRtimer = false;
      AppIn_G3CommonFlt = false;
      AppIn_G3DischargeFlt = false;
      AppIn_G4T1DischargeFlt = false;
      AppIn_G4T2DischargeFlt = false;
      AppIn_G4CommonFlt = false;
      AppIn_G4ChargeFlt = false;
      AppIn_OBCHeartbeatFail = false;
      AppIn_LoadVolt = 0;
      AppIn_PackVolt = 0;
      AppIn_ActiveDischg = Active_DisChrg_E.Inactive;
      AppIn_BattTemp = [26; 26; 26; 26; 26; 26;];
      AppIn_BattCurrent = 0;
      AppIn_BattVoltages = [4.2; 4.2; 4.2; 4.2; 4.2; 4.2; 4.2; 4.2; 4.2; 4.2; 4.2; 4.2; 4.2; 4.2; 4.2; 4.2; 4.2; 4.2; 4.2; 4.2];
      AppIn_LastStoredSOC = 0;
      AppIn_LastStoredCycle = 0;
      AppIn_I2Cerror = false;
      AppIn_LastStoredSOH = 0;
      AppIn_MachineStatus = VDU_MACHINE_STS_E.VDU_SLEEP;
      AppIn_HVMosfetfb = false;
      AppIn_DCDCMosfetfb = false;
      AppIn_PMosfetfb = false;
      AppIn_BMSVltSnsrFail = false;
      AppIn_BattPackTempSnsrFail = false;
      AppIn_VltImbFlt = false;
      AppIn_TempImbWarn = false;
      AppIn_EEPROMSoCWarn15 = false;
    state step_1
      AppIn_HardwiredIgn = true;
    state step_2
      AppIn_MCUHVIL  = true;
    state step_3
      AppIn_PMosfetfb = true;
    state step_4
      AppIn_LoadVolt = 72;
      AppIn_PackVolt = 75;
    state step_5
      AppIn_HVMosfetfb = true;
    state step_6
      AppIn_DCDCMosfetfb = true;
    state step_7
      AppIn_PMosfetfb = false;
    state step_8
    state step_9
      AppIn_G4T1DischargeFlt = true;
    state step_10
      AppIn_G4T2DischargeFlt = true;
    (default) -> G4T1DischgToG4T2Dischg.Run
    G4T1DischgToG4T2Dischg.Run -> G4T1DischgToG4T2Dischg.step_1
    G4T1DischgToG4T2Dischg.step_1 -> G4T1DischgToG4T2Dischg.step_2 : [ after(0.2,sec) ]
    G4T1DischgToG4T2Dischg.step_2 -> G4T1DischgToG4T2Dischg.step_3 : [ after(0.2,sec) ]
    G4T1DischgToG4T2Dischg.step_3 -> G4T1DischgToG4T2Dischg.step_4 : [ after(0.3,sec) ]
    G4T1DischgToG4T2Dischg.step_4 -> G4T1DischgToG4T2Dischg.step_5 : [ after(0.2,sec) ]
    G4T1DischgToG4T2Dischg.step_5 -> G4T1DischgToG4T2Dischg.step_6 : [ after(0.3,sec) ]
    G4T1DischgToG4T2Dischg.step_6 -> G4T1DischgToG4T2Dischg.step_7 : [ after(0.3,sec) ]
    G4T1DischgToG4T2Dischg.step_7 -> G4T1DischgToG4T2Dischg.step_8 : [ after(0.3,sec) ]
    G4T1DischgToG4T2Dischg.step_8 -> G4T1DischgToG4T2Dischg.step_9 : [ after(1,sec) ]
    G4T1DischgToG4T2Dischg.step_9 -> G4T1DischgToG4T2Dischg.step_10 : [ after(6,sec) ]
  state SleepToCharge
    state Run
      %% Initialize data outputs.
      AppIn_HardwiredIgn = false;
      AppIn_OBCwakeup = OBC_E.Wake_Up;
      AppIn_RTCwakeup = false;
      AppIn_MCUHVIL = false;
      AppIn_OBCHVIL = false;
      AppIn_SoCLEDSW = false;
      AppIn_ChgMode = Charger_Mode_E.OFF;
      AppIn_CVmodeTimer = CV_Mode_Timer_E.Off;
      AppIn_TRerror = false;
      AppIn_TRtimer = false;
      AppIn_G3CommonFlt = false;
      AppIn_G3DischargeFlt = false;
      AppIn_G4T1DischargeFlt = false;
      AppIn_G4T2DischargeFlt = false;
      AppIn_G4CommonFlt = false;
      AppIn_G4ChargeFlt = false;
      AppIn_OBCHeartbeatFail = true;
      AppIn_LoadVolt = 63;
      AppIn_PackVolt = 64;
      AppIn_ActiveDischg = Active_DisChrg_E.Inactive;
      AppIn_BattTemp = [26; 26; 26; 26; 26; 26;];
      AppIn_BattCurrent = 0;
      AppIn_BattVoltages = [4.2; 4.2; 4.2; 4.2; 4.2; 4.2; 4.2; 4.2; 4.2; 4.2; 4.2; 4.2; 4.2; 4.2; 4.2; 4.2; 4.2; 4.2; 4.2; 4.2];
      AppIn_LastStoredSOC = 0;
      AppIn_LastStoredCycle = 0;
      AppIn_I2Cerror = false;
      AppIn_LastStoredSOH = 0;
      AppIn_MachineStatus = VDU_MACHINE_STS_E.VDU_SLEEP;
      AppIn_HVMosfetfb = false;
      AppIn_DCDCMosfetfb = false;
      AppIn_PMosfetfb = false;
      AppIn_BMSVltSnsrFail = false;
      AppIn_BattPackTempSnsrFail = false;
      AppIn_VltImbFlt = false;
      AppIn_TempImbWarn = false;
      AppIn_EEPROMSoCWarn15 = false;
    state step_1
      AppIn_RTCwakeup = true;
    state step_4
      AppIn_OBCHVIL = false;
    state step_5
      AppIn_OBCwakeup = OBC_E.Sleep;
      AppIn_OBCHVIL = true;
    state step_6
      AppIn_OBCwakeup = OBC_E.Wake_Up;
    state step_7
      AppIn_ChgMode = Charger_Mode_E.Error;
      AppIn_OBCHeartbeatFail = false;
      AppIn_BattVoltages = [4.2; 4.2; 4.2; 4.2; 4.2; 2.0; 4.2; 4.2; 4.2; 4.2; 4.2; 4.2; 4.2; 4.2; 4.2; 4.2; 4.2; 4.2; 4.2; 4.2];
    state step_8
      AppIn_ChgMode = Charger_Mode_E.OFF;
    state step_2
      AppIn_BattVoltages = [4.2; 4.2; 4.2; 4.2; 4.2; 4.2; 4.2; 4.2; 4.2; 4.2; 4.2; 4.2; 4.2; 4.2; 4.2; 4.2; 4.2; 4.2; 4.2; 4.2];
      AppIn_RTCwakeup = false;
      state step_2_1
        AppIn_PMosfetfb = true;
      state step_2_2
        AppIn_HVMosfetfb = true;
      state step_2_3
        AppIn_PMosfetfb = false;
      (default) -> SleepToCharge.step_2.step_2_1
      SleepToCharge.step_2.step_2_1 -> SleepToCharge.step_2.step_2_2 : [ after(0.3,sec) ]
      SleepToCharge.step_2.step_2_2 -> SleepToCharge.step_2.step_2_3 : [ after(0.2,sec) ]
    state step_3
      AppIn_OBCHeartbeatFail = true;
      state step_3_1
        AppIn_HVMosfetfb = false;
      (default) -> SleepToCharge.step_3.step_3_1
    (default) -> SleepToCharge.Run
    SleepToCharge.Run -> SleepToCharge.step_1 : [ after(0.2,sec) ]
    SleepToCharge.step_1 -> SleepToCharge.step_4 : [ after(0.2,sec) ]
    SleepToCharge.step_4 -> SleepToCharge.step_5 : [ after(0.1,sec) ]
    SleepToCharge.step_5 -> SleepToCharge.step_6 : [ after(0.1,sec) ]
    SleepToCharge.step_6 -> SleepToCharge.step_7 : [ after(0.1,sec) ]
    SleepToCharge.step_7 -> SleepToCharge.step_8 : [ after(0.3,sec) ]
    SleepToCharge.step_8 -> SleepToCharge.step_2 : [ after(0.2,sec) ]
    SleepToCharge.step_2 -> SleepToCharge.step_3 : [ after(5,sec) ]
  state SleepToDischarge
    state Run
      %% Initialize data outputs.
      AppIn_HardwiredIgn = false;
      AppIn_OBCwakeup = OBC_E.Sleep;
      AppIn_RTCwakeup = false;
      AppIn_MCUHVIL = false;
      AppIn_OBCHVIL = false;
      AppIn_SoCLEDSW = false;
      AppIn_ChgMode = Charger_Mode_E.OFF;
      AppIn_CVmodeTimer = CV_Mode_Timer_E.Off;
      AppIn_TRerror = false;
      AppIn_TRtimer = false;
      AppIn_G3CommonFlt = false;
      AppIn_G3DischargeFlt = false;
      AppIn_G4T1DischargeFlt = false;
      AppIn_G4T2DischargeFlt = false;
      AppIn_G4CommonFlt = false;
      AppIn_G4ChargeFlt = false;
      AppIn_OBCHeartbeatFail = false;
      AppIn_LoadVolt = 63;
      AppIn_PackVolt = 64;
      AppIn_ActiveDischg = Active_DisChrg_E.Inactive;
      AppIn_BattTemp = [26; 26; 26; 26; 26; 26;];
      AppIn_BattCurrent = 0;
      AppIn_BattVoltages = [4.2; 4.2; 4.2; 4.2; 4.2; 4.2; 4.2; 4.2; 4.2; 4.2; 4.2; 4.2; 4.2; 4.2; 4.2; 4.2; 4.2; 4.2; 4.2; 4.2];
      AppIn_LastStoredSOC = 0;
      AppIn_LastStoredCycle = 0;
      AppIn_I2Cerror = false;
      AppIn_LastStoredSOH = 0;
      AppIn_MachineStatus = VDU_MACHINE_STS_E.VDU_SLEEP;
      AppIn_HVMosfetfb = false;
      AppIn_DCDCMosfetfb = false;
      AppIn_PMosfetfb = false;
      AppIn_BMSVltSnsrFail = false;
      AppIn_BattPackTempSnsrFail = false;
      AppIn_VltImbFlt = false;
      AppIn_TempImbWarn = false;
      AppIn_EEPROMSoCWarn15 = false;
    state step_4
      AppIn_OBCHeartbeatFail = true;
    state step_1
      AppIn_SoCLEDSW = true;
    state step_5
      AppIn_HardwiredIgn = true;
      AppIn_OBCHVIL = true;
    state step_6
      AppIn_OBCHVIL = false;
    state step_2
      AppIn_MCUHVIL = true;
      state step_2_1
        AppIn_PMosfetfb = true;
      state step_2_2
        AppIn_HVMosfetfb = true;
      state step_2_3
        AppIn_DCDCMosfetfb = true;
      state step_2_4
        AppIn_PMosfetfb = false;
      (default) -> SleepToDischarge.step_2.step_2_1
      SleepToDischarge.step_2.step_2_1 -> SleepToDischarge.step_2.step_2_2 : [ after(0.3,sec) ]
      SleepToDischarge.step_2.step_2_2 -> SleepToDischarge.step_2.step_2_3 : [ after(0.2,sec) ]
      SleepToDischarge.step_2.step_2_3 -> SleepToDischarge.step_2.step_2_4 : [ after(0.2,sec) ]
    state step_7
      AppIn_OBCwakeup = OBC_E.Wake_Up;
    state step_8
      AppIn_OBCHeartbeatFail = false;
    state step_3
      AppIn_HardwiredIgn = false;
      AppIn_OBCwakeup = OBC_E.Sleep;
      state step_3_1
        AppIn_HVMosfetfb = false;
      (default) -> SleepToDischarge.step_3.step_3_1
    (default) -> SleepToDischarge.Run
    SleepToDischarge.Run -> SleepToDischarge.step_4 : [ after(0.3,sec) ]
    SleepToDischarge.step_4 -> SleepToDischarge.step_1 : [ after(0.1,sec) ]
    SleepToDischarge.step_1 -> SleepToDischarge.step_5 : [ after(0.2,sec) ]
    SleepToDischarge.step_5 -> SleepToDischarge.step_6 : [ after(0.1,sec) ]
    SleepToDischarge.step_6 -> SleepToDischarge.step_2 : [ after(0.1,sec) ]
    SleepToDischarge.step_2 -> SleepToDischarge.step_7 : [ after(5,sec) ]
    SleepToDischarge.step_7 -> SleepToDischarge.step_8 : [ after(0.1,sec) ]
    SleepToDischarge.step_8 -> SleepToDischarge.step_3 : [ after(0.1,sec) ]
  state SleepToChgToSleep
    state Run
      %% Initialize data outputs.
      AppIn_HardwiredIgn = false;
      AppIn_OBCwakeup = OBC_E.Sleep;
      AppIn_RTCwakeup = false;
      AppIn_MCUHVIL = false;
      AppIn_OBCHVIL = true;
      AppIn_SoCLEDSW = false;
      AppIn_ChgMode = Charger_Mode_E.OFF;
      AppIn_CVmodeTimer = CV_Mode_Timer_E.Off;
      AppIn_TRerror = false;
      AppIn_TRtimer = false;
      AppIn_G3CommonFlt = false;
      AppIn_G3DischargeFlt = false;
      AppIn_G4T1DischargeFlt = false;
      AppIn_G4T2DischargeFlt = false;
      AppIn_G4CommonFlt = false;
      AppIn_G4ChargeFlt = false;
      AppIn_OBCHeartbeatFail = false;
      AppIn_LoadVolt = 63;
      AppIn_PackVolt = 84;
      AppIn_ActiveDischg = Active_DisChrg_E.Inactive;
      AppIn_BattTemp = [26; 26; 26; 26; 26; 26;];
      AppIn_BattCurrent = 0;
      AppIn_BattVoltages = [4.2; 4.2; 4.2; 4.2; 4.2; 4.2; 4.2; 4.2; 4.2; 4.2; 4.2; 4.2; 4.2; 4.2; 4.2; 4.2; 4.2; 4.2; 4.2; 4.2];
      AppIn_LastStoredSOC = 0;
      AppIn_LastStoredCycle = 0;
      AppIn_I2Cerror = false;
      AppIn_LastStoredSOH = 0;
      AppIn_MachineStatus = VDU_MACHINE_STS_E.VDU_SLEEP;
      AppIn_HVMosfetfb = false;
      AppIn_DCDCMosfetfb = false;
      AppIn_PMosfetfb = false;
      AppIn_BMSVltSnsrFail = false;
      AppIn_BattPackTempSnsrFail = false;
      AppIn_VltImbFlt = false;
      AppIn_TempImbWarn = false;
      AppIn_EEPROMSoCWarn15 = false;
    state step_7
      AppIn_OBCwakeup = OBC_E.Wake_Up;
    state step_1
      AppIn_LoadVolt = 63;
      AppIn_PackVolt = 64;
    state step_2
    state step_3
      AppIn_RTCwakeup = true;
      state step_3_1
        AppIn_PMosfetfb = true;
      state step_3_2
        AppIn_HVMosfetfb = true;
      state step_3_3
        AppIn_PMosfetfb = false;
      (default) -> SleepToChgToSleep.step_3.step_3_1
      SleepToChgToSleep.step_3.step_3_2 -> SleepToChgToSleep.step_3.step_3_3 : [ after(0.2,sec) ]
      SleepToChgToSleep.step_3.step_3_1 -> SleepToChgToSleep.step_3.step_3_2 : [ after(0.3,sec) ]
    state step_4
      AppIn_ChgMode = Charger_Mode_E.Error;
      state step_4_1
        AppIn_HVMosfetfb = false;
      (default) -> SleepToChgToSleep.step_4.step_4_1
    state step_5
      AppIn_OBCwakeup = OBC_E.Sleep;
      AppIn_RTCwakeup = true;
      AppIn_ChgMode = Charger_Mode_E.OFF;
    state step_6
    (default) -> SleepToChgToSleep.Run
    SleepToChgToSleep.Run -> SleepToChgToSleep.step_7 : [ after(0.1,sec) ]
    SleepToChgToSleep.step_1 -> SleepToChgToSleep.step_2 : [ after(9,sec) ]
    SleepToChgToSleep.step_2 -> SleepToChgToSleep.step_3 : [ after(3,sec) ]
    SleepToChgToSleep.step_3 -> SleepToChgToSleep.step_4 : [ after(1,sec) ]
    SleepToChgToSleep.step_4 -> SleepToChgToSleep.step_5 : [ after(1,sec) ]
    SleepToChgToSleep.step_5 -> SleepToChgToSleep.step_6 : [ after(9.1,sec) ]
    SleepToChgToSleep.step_7 -> SleepToChgToSleep.step_1 : [ after(0.1,sec) ]
  state SleepToChg
    state Run
      %% Initialize data outputs.
      AppIn_HardwiredIgn = false;
      AppIn_OBCwakeup = OBC_E.Sleep;
      AppIn_RTCwakeup = false;
      AppIn_MCUHVIL = false;
      AppIn_OBCHVIL = false;
      AppIn_SoCLEDSW = false;
      AppIn_ChgMode = Charger_Mode_E.OFF;
      AppIn_CVmodeTimer = CV_Mode_Timer_E.Off;
      AppIn_TRerror = false;
      AppIn_TRtimer = false;
      AppIn_G3CommonFlt = false;
      AppIn_G3DischargeFlt = false;
      AppIn_G4T1DischargeFlt = false;
      AppIn_G4T2DischargeFlt = false;
      AppIn_G4CommonFlt = false;
      AppIn_G4ChargeFlt = false;
      AppIn_OBCHeartbeatFail = false;
      AppIn_LoadVolt = 63;
      AppIn_PackVolt = 64;
      AppIn_ActiveDischg = Active_DisChrg_E.Inactive;
      AppIn_BattTemp = [26; 26; 26; 26; 26; 26;];
      AppIn_BattCurrent = 0;
      AppIn_BattVoltages = [4.2; 4.2; 4.2; 4.2; 4.2; 4.2; 4.2; 4.2; 4.2; 4.2; 4.2; 4.2; 4.2; 4.2; 4.2; 4.2; 4.2; 4.2; 4.2; 4.2];
      AppIn_LastStoredSOC = 0;
      AppIn_LastStoredCycle = 0;
      AppIn_I2Cerror = false;
      AppIn_LastStoredSOH = 0;
      AppIn_MachineStatus = VDU_MACHINE_STS_E.VDU_SLEEP;
      AppIn_HVMosfetfb = false;
      AppIn_DCDCMosfetfb = false;
      AppIn_PMosfetfb = false;
      AppIn_BMSVltSnsrFail = false;
      AppIn_BattPackTempSnsrFail = false;
      AppIn_VltImbFlt = false;
      AppIn_TempImbWarn = false;
      AppIn_EEPROMSoCWarn15 = false;
    state step_1
      AppIn_HardwiredIgn = true;
    state step_2
      AppIn_OBCwakeup = OBC_E.Wake_Up;
      AppIn_OBCHVIL = true;
      state step_2_1
        AppIn_PMosfetfb = true;
      state step_2_2
        AppIn_HVMosfetfb = true;
      state step_2_3
        AppIn_PMosfetfb = false;
      (default) -> SleepToChg.step_2.step_2_1
      SleepToChg.step_2.step_2_1 -> SleepToChg.step_2.step_2_2 : [ after(0.3,sec) ]
      SleepToChg.step_2.step_2_2 -> SleepToChg.step_2.step_2_3 : [ after(0.2,sec) ]
    state step_3
      AppIn_CVmodeTimer = CV_Mode_Timer_E.Expired;
      AppIn_OBCwakeup = OBC_E.Sleep;
      state step_3_1
        AppIn_HVMosfetfb = false;
      (default) -> SleepToChg.step_3.step_3_1
    state step_4
      AppIn_HardwiredIgn = false;
    (default) -> SleepToChg.Run
    SleepToChg.Run -> SleepToChg.step_1 : [ after(0.2,sec) ]
    SleepToChg.step_1 -> SleepToChg.step_2 : [ after(0.2,sec) ]
    SleepToChg.step_2 -> SleepToChg.step_3 : [ after(5,sec) ]
    SleepToChg.step_3 -> SleepToChg.step_4 : [ after(5,sec) ]
  state SleepToChrg
    state Run
      %% Initialize data outputs.
      AppIn_HardwiredIgn = false;
      AppIn_OBCwakeup = OBC_E.Sleep;
      AppIn_RTCwakeup = false;
      AppIn_MCUHVIL = false;
      AppIn_OBCHVIL = false;
      AppIn_SoCLEDSW = false;
      AppIn_ChgMode = Charger_Mode_E.OFF;
      AppIn_CVmodeTimer = CV_Mode_Timer_E.Off;
      AppIn_TRerror = false;
      AppIn_TRtimer = false;
      AppIn_G3CommonFlt = false;
      AppIn_G3DischargeFlt = false;
      AppIn_G4T1DischargeFlt = false;
      AppIn_G4T2DischargeFlt = false;
      AppIn_G4CommonFlt = false;
      AppIn_G4ChargeFlt = false;
      AppIn_OBCHeartbeatFail = false;
      AppIn_LoadVolt = 63;
      AppIn_PackVolt = 64;
      AppIn_ActiveDischg = Active_DisChrg_E.Inactive;
      AppIn_BattTemp = [26; 26; 26; 26; 26; 26;];
      AppIn_BattCurrent = 0;
      AppIn_BattVoltages = [4.2; 4.2; 4.2; 4.2; 4.2; 4.2; 4.2; 4.2; 4.2; 4.2; 4.2; 4.2; 4.2; 4.2; 4.2; 4.2; 4.2; 4.2; 4.2; 4.2];
      AppIn_LastStoredSOC = 0;
      AppIn_LastStoredCycle = 0;
      AppIn_I2Cerror = false;
      AppIn_LastStoredSOH = 0;
      AppIn_MachineStatus = VDU_MACHINE_STS_E.VDU_SLEEP;
      AppIn_HVMosfetfb = false;
      AppIn_DCDCMosfetfb = false;
      AppIn_PMosfetfb = false;
      AppIn_BMSVltSnsrFail = false;
      AppIn_BattPackTempSnsrFail = false;
      AppIn_VltImbFlt = false;
      AppIn_TempImbWarn = false;
      AppIn_EEPROMSoCWarn15 = false;
    state step_1
      AppIn_HardwiredIgn = true;
    state step_2
      AppIn_OBCwakeup = OBC_E.Wake_Up;
      AppIn_OBCHVIL = true;
      state step_2_1
        AppIn_PMosfetfb = true;
      state step_2_2
        AppIn_HVMosfetfb = true;
      state step_2_3
        AppIn_PMosfetfb = false;
      (default) -> SleepToChrg.step_2.step_2_1
      SleepToChrg.step_2.step_2_1 -> SleepToChrg.step_2.step_2_2 : [ after(0.3,sec) ]
      SleepToChrg.step_2.step_2_2 -> SleepToChrg.step_2.step_2_3 : [ after(0.2,sec) ]
    state step_3
      AppIn_OBCHVIL = false;
      AppIn_OBCwakeup = OBC_E.Sleep;
      state step_3_1
        AppIn_HVMosfetfb = false;
      (default) -> SleepToChrg.step_3.step_3_1
    state step_4
      AppIn_HardwiredIgn = false;
    (default) -> SleepToChrg.Run
    SleepToChrg.Run -> SleepToChrg.step_1 : [ after(0.2,sec) ]
    SleepToChrg.step_1 -> SleepToChrg.step_2 : [ after(0.2,sec) ]
    SleepToChrg.step_2 -> SleepToChrg.step_3 : [ after(5,sec) ]
    SleepToChrg.step_3 -> SleepToChrg.step_4 : [ after(5,sec) ]
  state SleepToStbToG3CommFlt
    state Run
      %% Initialize data outputs.
      AppIn_HardwiredIgn = false;
      AppIn_OBCwakeup = OBC_E.Sleep;
      AppIn_RTCwakeup = false;
      AppIn_MCUHVIL = false;
      AppIn_OBCHVIL = false;
      AppIn_SoCLEDSW = false;
      AppIn_ChgMode = Charger_Mode_E.OFF;
      AppIn_CVmodeTimer = CV_Mode_Timer_E.Off;
      AppIn_TRerror = false;
      AppIn_TRtimer = false;
      AppIn_G3CommonFlt = false;
      AppIn_G3DischargeFlt = false;
      AppIn_G4T1DischargeFlt = false;
      AppIn_G4T2DischargeFlt = false;
      AppIn_G4CommonFlt = false;
      AppIn_G4ChargeFlt = false;
      AppIn_OBCHeartbeatFail = false;
      AppIn_LoadVolt = 63;
      AppIn_PackVolt = 64;
      AppIn_ActiveDischg = Active_DisChrg_E.Inactive;
      AppIn_BattTemp = [26; 26; 26; 26; 26; 26;];
      AppIn_BattCurrent = 0;
      AppIn_BattVoltages = [4.2; 4.2; 4.2; 4.2; 4.2; 4.2; 4.2; 4.2; 4.2; 4.2; 4.2; 4.2; 4.2; 4.2; 4.2; 4.2; 4.2; 4.2; 4.2; 4.2];
      AppIn_LastStoredSOC = 0;
      AppIn_LastStoredCycle = 0;
      AppIn_I2Cerror = false;
      AppIn_LastStoredSOH = 0;
      AppIn_MachineStatus = VDU_MACHINE_STS_E.VDU_SLEEP;
      AppIn_HVMosfetfb = false;
      AppIn_DCDCMosfetfb = false;
      AppIn_PMosfetfb = false;
      AppIn_BMSVltSnsrFail = false;
      AppIn_BattPackTempSnsrFail = false;
      AppIn_VltImbFlt = false;
      AppIn_TempImbWarn = false;
      AppIn_EEPROMSoCWarn15 = false;
    state step_1
      AppIn_HardwiredIgn = true;
    state step_2
      AppIn_G3CommonFlt = true;
    state step_3
      state step_3_1
      state step_3_2
        AppIn_HardwiredIgn = false;
      state step_3_3
        AppIn_TRerror = true;
      state step_3_4
        AppIn_TRerror = false;
      (default) -> SleepToStbToG3CommFlt.step_3.step_3_1
      SleepToStbToG3CommFlt.step_3.step_3_1 -> SleepToStbToG3CommFlt.step_3.step_3_2 : [ after(0.1,sec) ]
      SleepToStbToG3CommFlt.step_3.step_3_2 -> SleepToStbToG3CommFlt.step_3.step_3_3 : [ after(0.2,sec) ]
      SleepToStbToG3CommFlt.step_3.step_3_3 -> step_3_4 : [ after(0.2,sec) ]
    (default) -> SleepToStbToG3CommFlt.Run
    SleepToStbToG3CommFlt.Run -> SleepToStbToG3CommFlt.step_1
    SleepToStbToG3CommFlt.step_1 -> SleepToStbToG3CommFlt.step_2 : [ after(0.2,sec) ]
    SleepToStbToG3CommFlt.step_2 -> SleepToStbToG3CommFlt.step_3 : [ after(0.2,sec) ]
  state SleepToStbToG4CommFlt
    state Run
      %% Initialize data outputs.
      AppIn_HardwiredIgn = false;
      AppIn_OBCwakeup = OBC_E.Sleep;
      AppIn_RTCwakeup = false;
      AppIn_MCUHVIL = false;
      AppIn_OBCHVIL = false;
      AppIn_SoCLEDSW = false;
      AppIn_ChgMode = Charger_Mode_E.OFF;
      AppIn_CVmodeTimer = CV_Mode_Timer_E.Off;
      AppIn_TRerror = false;
      AppIn_TRtimer = false;
      AppIn_G3CommonFlt = false;
      AppIn_G3DischargeFlt = false;
      AppIn_G4T1DischargeFlt = false;
      AppIn_G4T2DischargeFlt = false;
      AppIn_G4CommonFlt = false;
      AppIn_G4ChargeFlt = false;
      AppIn_OBCHeartbeatFail = false;
      AppIn_LoadVolt = 63;
      AppIn_PackVolt = 64;
      AppIn_ActiveDischg = Active_DisChrg_E.Inactive;
      AppIn_BattTemp = [26; 26; 26; 26; 26; 26;];
      AppIn_BattCurrent = 0;
      AppIn_BattVoltages = [4.2; 4.2; 4.2; 4.2; 4.2; 4.2; 4.2; 4.2; 4.2; 4.2; 4.2; 4.2; 4.2; 4.2; 4.2; 4.2; 4.2; 4.2; 4.2; 4.2];
      AppIn_LastStoredSOC = 0;
      AppIn_LastStoredCycle = 0;
      AppIn_I2Cerror = false;
      AppIn_LastStoredSOH = 0;
      AppIn_MachineStatus = VDU_MACHINE_STS_E.VDU_SLEEP;
      AppIn_HVMosfetfb = false;
      AppIn_DCDCMosfetfb = false;
      AppIn_PMosfetfb = false;
      AppIn_BMSVltSnsrFail = false;
      AppIn_BattPackTempSnsrFail = false;
      AppIn_VltImbFlt = false;
      AppIn_TempImbWarn = false;
      AppIn_EEPROMSoCWarn15 = false;
    state step_1
      AppIn_HardwiredIgn = true;
    state step_2
      AppIn_G4CommonFlt = true;
    state step_3
      AppIn_HardwiredIgn = false;
      AppIn_TRerror = true;
      AppIn_TRtimer = true;
    (default) -> SleepToStbToG4CommFlt.Run
    SleepToStbToG4CommFlt.Run -> SleepToStbToG4CommFlt.step_1
    SleepToStbToG4CommFlt.step_1 -> SleepToStbToG4CommFlt.step_2 : [ after(0.2,sec) ]
    SleepToStbToG4CommFlt.step_2 -> SleepToStbToG4CommFlt.step_3 : [ after(0.7,sec) ]
  state SleepToStbToG4CommFlt1
    state Run
      %% Initialize data outputs.
      AppIn_HardwiredIgn = false;
      AppIn_OBCwakeup = OBC_E.Sleep;
      AppIn_RTCwakeup = false;
      AppIn_MCUHVIL = false;
      AppIn_OBCHVIL = false;
      AppIn_SoCLEDSW = false;
      AppIn_ChgMode = Charger_Mode_E.OFF;
      AppIn_CVmodeTimer = CV_Mode_Timer_E.Off;
      AppIn_TRerror = false;
      AppIn_TRtimer = false;
      AppIn_G3CommonFlt = false;
      AppIn_G3DischargeFlt = false;
      AppIn_G4T1DischargeFlt = false;
      AppIn_G4T2DischargeFlt = false;
      AppIn_G4CommonFlt = false;
      AppIn_G4ChargeFlt = false;
      AppIn_OBCHeartbeatFail = false;
      AppIn_LoadVolt = 63;
      AppIn_PackVolt = 64;
      AppIn_ActiveDischg = Active_DisChrg_E.Inactive;
      AppIn_BattTemp = [26; 26; 26; 26; 26; 26;];
      AppIn_BattCurrent = 0;
      AppIn_BattVoltages = [4.2; 4.2; 4.2; 4.2; 4.2; 4.2; 4.2; 4.2; 4.2; 4.2; 4.2; 4.2; 4.2; 4.2; 4.2; 4.2; 4.2; 4.2; 4.2; 4.2];
      AppIn_LastStoredSOC = 0;
      AppIn_LastStoredCycle = 0;
      AppIn_I2Cerror = false;
      AppIn_LastStoredSOH = 0;
      AppIn_MachineStatus = VDU_MACHINE_STS_E.VDU_SLEEP;
      AppIn_HVMosfetfb = false;
      AppIn_DCDCMosfetfb = false;
      AppIn_PMosfetfb = false;
      AppIn_BMSVltSnsrFail = false;
      AppIn_BattPackTempSnsrFail = false;
      AppIn_VltImbFlt = false;
      AppIn_TempImbWarn = false;
      AppIn_EEPROMSoCWarn15 = false;
    state step_1
      AppIn_HardwiredIgn = true;
    state step_2
      AppIn_G4CommonFlt = true;
    state step_3
      AppIn_HardwiredIgn = false;
      AppIn_G4CommonFlt = false;
    (default) -> SleepToStbToG4CommFlt1.Run
    SleepToStbToG4CommFlt1.Run -> SleepToStbToG4CommFlt1.step_1
    SleepToStbToG4CommFlt1.step_1 -> SleepToStbToG4CommFlt1.step_2 : [ after(0.2,sec) ]
    SleepToStbToG4CommFlt1.step_2 -> SleepToStbToG4CommFlt1.step_3 : [ after(0.7,sec) ]
  state SleepToDischgToFlt
    state Run
      %% Initialize data outputs.
      AppIn_HardwiredIgn = false;
      AppIn_OBCwakeup = OBC_E.Sleep;
      AppIn_RTCwakeup = false;
      AppIn_MCUHVIL = false;
      AppIn_OBCHVIL = false;
      AppIn_SoCLEDSW = false;
      AppIn_ChgMode = Charger_Mode_E.OFF;
      AppIn_CVmodeTimer = CV_Mode_Timer_E.Off;
      AppIn_TRerror = false;
      AppIn_TRtimer = false;
      AppIn_G3CommonFlt = false;
      AppIn_G3DischargeFlt = false;
      AppIn_G4T1DischargeFlt = false;
      AppIn_G4T2DischargeFlt = false;
      AppIn_G4CommonFlt = false;
      AppIn_G4ChargeFlt = false;
      AppIn_OBCHeartbeatFail = false;
      AppIn_LoadVolt = 63;
      AppIn_PackVolt = 64;
      AppIn_ActiveDischg = Active_DisChrg_E.Inactive;
      AppIn_BattTemp = [26; 26; 26; 26; 26; 26;];
      AppIn_BattCurrent = 0;
      AppIn_BattVoltages = [4.2; 4.2; 4.2; 4.2; 4.2; 4.2; 4.2; 4.2; 4.2; 4.2; 4.2; 4.2; 4.2; 4.2; 4.2; 4.2; 4.2; 4.2; 4.2; 4.2];
      AppIn_LastStoredSOC = 0;
      AppIn_LastStoredCycle = 0;
      AppIn_I2Cerror = false;
      AppIn_LastStoredSOH = 0;
      AppIn_MachineStatus = VDU_MACHINE_STS_E.VDU_SLEEP;
      AppIn_HVMosfetfb = false;
      AppIn_DCDCMosfetfb = false;
      AppIn_PMosfetfb = false;
      AppIn_BMSVltSnsrFail = false;
      AppIn_BattPackTempSnsrFail = false;
      AppIn_VltImbFlt = false;
      AppIn_TempImbWarn = false;
      AppIn_EEPROMSoCWarn15 = false;
    state step_1
      AppIn_HardwiredIgn = true;
    state step_2
      AppIn_MCUHVIL = true;
      state step_2_1
        AppIn_PMosfetfb = true;
      state step_2_2
        AppIn_HVMosfetfb = true;
      state step_2_3
        AppIn_DCDCMosfetfb = true;
      state step_2_4
        AppIn_PMosfetfb = false;
      (default) -> SleepToDischgToFlt.step_2.step_2_1
      SleepToDischgToFlt.step_2.step_2_1 -> SleepToDischgToFlt.step_2.step_2_2 : [ after(0.2,sec) ]
      SleepToDischgToFlt.step_2.step_2_2 -> SleepToDischgToFlt.step_2.step_2_3 : [ after(0.2,sec) ]
      SleepToDischgToFlt.step_2.step_2_3 -> SleepToDischgToFlt.step_2.step_2_4 : [ after(0.2,sec) ]
    state step_3
      AppIn_G4T1DischargeFlt = true;
    state step_4
      AppIn_G4T1DischargeFlt = false;
      state step_4_1
        AppIn_PMosfetfb = true;
      state step_4_2
        AppIn_HVMosfetfb = true;
      state step_4_3
        AppIn_DCDCMosfetfb = true;
      state step_4_4
        AppIn_PMosfetfb = false;
      (default) -> SleepToDischgToFlt.step_4.step_4_1
      SleepToDischgToFlt.step_4.step_4_1 -> SleepToDischgToFlt.step_4.step_4_2 : [ after(0.2,sec) ]
      SleepToDischgToFlt.step_4.step_4_2 -> SleepToDischgToFlt.step_4.step_4_3 : [ after(0.2,sec) ]
      SleepToDischgToFlt.step_4.step_4_3 -> SleepToDischgToFlt.step_4.step_4_4 : [ after(0.2,sec) ]
    state step_5
      AppIn_HardwiredIgn = false;
      state step_5_1
        AppIn_HVMosfetfb = false;
      (default) -> SleepToDischgToFlt.step_5.step_5_1
    (default) -> SleepToDischgToFlt.Run
    SleepToDischgToFlt.Run -> SleepToDischgToFlt.step_1
    SleepToDischgToFlt.step_1 -> SleepToDischgToFlt.step_2 : [ after(0.2,sec) ]
    SleepToDischgToFlt.step_2 -> SleepToDischgToFlt.step_3 : [ after(2,sec) ]
    SleepToDischgToFlt.step_3 -> SleepToDischgToFlt.step_4 : [ after(6,sec) ]
    SleepToDischgToFlt.step_4 -> SleepToDischgToFlt.step_5 : [ after(2,sec) ]
  state SleepToDischgToFlt1
    state Run
      %% Initialize data outputs.
      AppIn_HardwiredIgn = false;
      AppIn_OBCwakeup = OBC_E.Sleep;
      AppIn_RTCwakeup = false;
      AppIn_MCUHVIL = false;
      AppIn_OBCHVIL = false;
      AppIn_SoCLEDSW = false;
      AppIn_ChgMode = Charger_Mode_E.OFF;
      AppIn_CVmodeTimer = CV_Mode_Timer_E.Off;
      AppIn_TRerror = false;
      AppIn_TRtimer = false;
      AppIn_G3CommonFlt = false;
      AppIn_G3DischargeFlt = false;
      AppIn_G4T1DischargeFlt = false;
      AppIn_G4T2DischargeFlt = false;
      AppIn_G4CommonFlt = false;
      AppIn_G4ChargeFlt = false;
      AppIn_OBCHeartbeatFail = false;
      AppIn_LoadVolt = 63;
      AppIn_PackVolt = 64;
      AppIn_ActiveDischg = Active_DisChrg_E.Inactive;
      AppIn_BattTemp = [26; 26; 26; 26; 26; 26;];
      AppIn_BattCurrent = 0;
      AppIn_BattVoltages = [4.2; 4.2; 4.2; 4.2; 4.2; 4.2; 4.2; 4.2; 4.2; 4.2; 4.2; 4.2; 4.2; 4.2; 4.2; 4.2; 4.2; 4.2; 4.2; 4.2];
      AppIn_LastStoredSOC = 0;
      AppIn_LastStoredCycle = 0;
      AppIn_I2Cerror = false;
      AppIn_LastStoredSOH = 0;
      AppIn_MachineStatus = VDU_MACHINE_STS_E.VDU_SLEEP;
      AppIn_HVMosfetfb = false;
      AppIn_DCDCMosfetfb = false;
      AppIn_PMosfetfb = false;
      AppIn_BMSVltSnsrFail = false;
      AppIn_BattPackTempSnsrFail = false;
      AppIn_VltImbFlt = false;
      AppIn_TempImbWarn = false;
      AppIn_EEPROMSoCWarn15 = false;
    state step_1
      AppIn_HardwiredIgn = true;
    state step_2
      AppIn_MCUHVIL = true;
      state step_2_1
        AppIn_PMosfetfb = true;
      state step_2_2
        AppIn_HVMosfetfb = true;
      state step_2_3
        AppIn_DCDCMosfetfb = true;
      state step_2_4
        AppIn_PMosfetfb = false;
      (default) -> SleepToDischgToFlt1.step_2.step_2_1
      SleepToDischgToFlt1.step_2.step_2_1 -> SleepToDischgToFlt1.step_2.step_2_2 : [ after(0.2,sec) ]
      SleepToDischgToFlt1.step_2.step_2_2 -> SleepToDischgToFlt1.step_2.step_2_3 : [ after(0.2,sec) ]
      SleepToDischgToFlt1.step_2.step_2_3 -> SleepToDischgToFlt1.step_2.step_2_4 : [ after(0.2,sec) ]
    state step_3
      AppIn_G3DischargeFlt = true;
    state step_4
      AppIn_G3DischargeFlt = false;
      state step_4_1
        AppIn_PMosfetfb = true;
      state step_4_2
        AppIn_HVMosfetfb = true;
      state step_4_3
        AppIn_DCDCMosfetfb = true;
      state step_4_4
        AppIn_PMosfetfb = false;
      (default) -> SleepToDischgToFlt1.step_4.step_4_1
      SleepToDischgToFlt1.step_4.step_4_1 -> SleepToDischgToFlt1.step_4.step_4_2 : [ after(0.2,sec) ]
      SleepToDischgToFlt1.step_4.step_4_2 -> SleepToDischgToFlt1.step_4.step_4_3 : [ after(0.2,sec) ]
      SleepToDischgToFlt1.step_4.step_4_3 -> SleepToDischgToFlt1.step_4.step_4_4 : [ after(0.2,sec) ]
    state step_5
      AppIn_HardwiredIgn = false;
      state step_5_1
        AppIn_HVMosfetfb = false;
      (default) -> SleepToDischgToFlt1.step_5.step_5_1
    (default) -> SleepToDischgToFlt1.Run
    SleepToDischgToFlt1.Run -> SleepToDischgToFlt1.step_1
    SleepToDischgToFlt1.step_1 -> SleepToDischgToFlt1.step_2 : [ after(0.2,sec) ]
    SleepToDischgToFlt1.step_2 -> SleepToDischgToFlt1.step_3 : [ after(2,sec) ]
    SleepToDischgToFlt1.step_3 -> SleepToDischgToFlt1.step_4 : [ after(6,sec) ]
    SleepToDischgToFlt1.step_4 -> SleepToDischgToFlt1.step_5 : [ after(2,sec) ]
  state SleepToDischgToFlt2
    state Run
      %% Initialize data outputs.
      AppIn_HardwiredIgn = false;
      AppIn_OBCwakeup = OBC_E.Sleep;
      AppIn_RTCwakeup = false;
      AppIn_MCUHVIL = false;
      AppIn_OBCHVIL = false;
      AppIn_SoCLEDSW = false;
      AppIn_ChgMode = Charger_Mode_E.OFF;
      AppIn_CVmodeTimer = CV_Mode_Timer_E.Off;
      AppIn_TRerror = false;
      AppIn_TRtimer = false;
      AppIn_G3CommonFlt = false;
      AppIn_G3DischargeFlt = false;
      AppIn_G4T1DischargeFlt = false;
      AppIn_G4T2DischargeFlt = false;
      AppIn_G4CommonFlt = false;
      AppIn_G4ChargeFlt = false;
      AppIn_OBCHeartbeatFail = false;
      AppIn_LoadVolt = 63;
      AppIn_PackVolt = 64;
      AppIn_ActiveDischg = Active_DisChrg_E.Inactive;
      AppIn_BattTemp = [26; 26; 26; 26; 26; 26;];
      AppIn_BattCurrent = 0;
      AppIn_BattVoltages = [4.2; 4.2; 4.2; 4.2; 4.2; 4.2; 4.2; 4.2; 4.2; 4.2; 4.2; 4.2; 4.2; 4.2; 4.2; 4.2; 4.2; 4.2; 4.2; 4.2];
      AppIn_LastStoredSOC = 0;
      AppIn_LastStoredCycle = 0;
      AppIn_I2Cerror = false;
      AppIn_LastStoredSOH = 0;
      AppIn_MachineStatus = VDU_MACHINE_STS_E.VDU_SLEEP;
      AppIn_HVMosfetfb = false;
      AppIn_DCDCMosfetfb = false;
      AppIn_PMosfetfb = false;
      AppIn_BMSVltSnsrFail = false;
      AppIn_BattPackTempSnsrFail = false;
      AppIn_VltImbFlt = false;
      AppIn_TempImbWarn = false;
      AppIn_EEPROMSoCWarn15 = false;
    state step_1
      AppIn_HardwiredIgn = true;
    state step_2
      AppIn_MCUHVIL = true;
      state step_2_1
        AppIn_PMosfetfb = true;
      state step_2_2
        AppIn_HVMosfetfb = true;
      state step_2_3
        AppIn_DCDCMosfetfb = true;
      state step_2_4
        AppIn_PMosfetfb = false;
      (default) -> SleepToDischgToFlt2.step_2.step_2_1
      SleepToDischgToFlt2.step_2.step_2_1 -> SleepToDischgToFlt2.step_2.step_2_2 : [ after(0.2,sec) ]
      SleepToDischgToFlt2.step_2.step_2_2 -> SleepToDischgToFlt2.step_2.step_2_3 : [ after(0.2,sec) ]
      SleepToDischgToFlt2.step_2.step_2_3 -> SleepToDischgToFlt2.step_2.step_2_4 : [ after(0.2,sec) ]
    state step_3
      AppIn_G3CommonFlt = true;
    state step_6
      AppIn_OBCHVIL = true;
    state step_4
      AppIn_OBCHVIL = false;
